simulink model "ASM_Traffic_new"  (R2024a)
settings: Solver=ode1  StartTime=SIM.tstart.v  StopTime=SIM.tend.v  FixedStep=SIM.StepSize.v  RelTol=1e-3
PostLoadFcn:
  | if any(exist('dsrtsu_mdlpostloadfcn', 'file') ~= 0), dsrtsu_mdlpostloadfcn('Execute', bdroot); end
  | try, asm_mdl_postloadfcn(bdroot, 'UpdateModel', 3600); catch, disp(lasterr); end,
InitFcn:
  | , if any(exist('rtifpga_mdlclblib', 'file') ~= 0), rtifpga_mdlclblib('Init', bdroot); end,
  | , if any(exist('dsmpb_private', 'file') ~= 0), dsmpb_private('dsmpb_mdlclblib', 'Init', bdroot); end,
undefined symbols (not defined in the file): _to_, a0b2, ASM_BrakeHydraulics_DemoSystems, ASM_VehicleDynamics_DemoSystems, b98103fe8ad365046cd0, BrakeCircuit, CPT, Crankshaft, DiscIntNeverNeededParam, dsmsi, FinalDriveAssembly, MDL, ModeSignals, Pos_BrakePedal_Maneuver, rad, RefSignals, s_to_rpm, SIM, SoftECU, Suspension, Tire, Transmission
libraries: ASM_Traffic_lib x135, simulink x100, ASM_Utils_lib x77, ASM_VehicleDynamics_lib x70, ASM_Environment_lib x22, dsmpblib x20, dsmsilib x15, MDLD_Utils_lib x10, ASM_BrakeHydraulics_lib x3
(part 27 of 63)

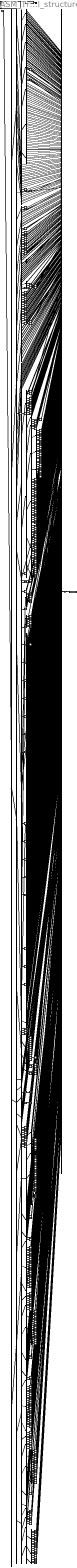
== system ASM_Traffic_new/Environment/SignalInterface/ASMSignalInterface/signal_structure ==
  ASMSignalBus : Inport
  Ambient : BusSelector  OutputSignals=T_Ambient[degC],p_Ambient[Pa]
  Angle_Fellows[x;y;z][deg] : BusSelector  OutputSignals=Angle_Roll_Fellows[deg],Angle_Pitch_Fellows[deg],Angle_Yaw_Fellows[deg],Angle_Wheel_Fellows[deg]
  BusSelector_1 : BusSelector  OutputSignals=Maneuver,Road,Traffic,GroundTruth,Sensors
  Collision_Sensor : BusSelector  OutputSignals=Collision_Sensor_1
  Collision_Sensor_1 : BusSelector  OutputSignals=Info,SensorOutput
  Common : BusSelector  OutputSignals=LaneID_PrefLane[],LaneID_Absolute[],LaneDirection_Absolute[],LaneDirection_Relative[],LaneWidth[m],LaneCurvature[1|m],Curvature[1|m]
  ContentID : Constant  Value=546881520
  Control : BusSelector  OutputSignals=Quadrant_Def_Mode[1Internal|2External],Quadrant_Dim_x[m],Quadrant_Dim_y[m],Interface_Mode[0Off|1ObjOnly|2ObjAndLanes],Interface_Init[0Off|1On],Interface_Init_Ready[0Off|1On]
  Control1 : BusSelector  OutputSignals=Quadrant_Def_Mode[1Internal|2External],Quadrant_Dim_x[m],Quadrant_Dim_y[m],Interface_Mode[0Off|1ObjOnly|2ObjAndLanes],Interface_Init[0Off|1On],Interface_Init_Ready[0Off|1On]
  CurrentLane : BusSelector  OutputSignals=Common,LeftSide,RightSide
  CustomPoints : BusSelector  OutputSignals=ID[],Object_ID[],Dist_CoorSys_S[m],Angle_Hor_CoorSys_S[deg],Pos_CoorSys_E[x;y;z][m]
  CustomPoints1 : BusSelector  OutputSignals=ID[],Object_ID[],Dist_CoorSys_S[m],Angle_Hor_CoorSys_S[deg],Pos_CoorSys_E[x;y;z][m]
  Data : BusSelector  OutputSignals=GroundTruth_Interface_Data[],HostVehicle_Data
  DataTypeConversion_{102,155..157,188,220,310..311,587,591..592,595..596,604..605} (15 alike) : DataTypeConversion  OutDataTypeStr=double
  Data_Access : BusSelector  OutputSignals=Num_MovObj[],Num_MovObj_in_GT_Area[],Num_StatObj[],Num_StatObj_in_GT_Area[],Num_Laneboundaries[],Num_Lanes[],Num_TrfLights[],Num_TrfLights_in_GT_Area[],Num_TrfSigns[],Num_TrfSigns_in_GT_Area[]
  DiscreteObjects : BusSelector  OutputSignals=Flag_DiscreteObject_Init_Ready[0|1],DiscreteObjectsState[],Data_Valid[],DiscreteObject_Data[]
  Dist_Response_Maneuver : BusSelector  OutputSignals=Distance_xy[m],Distance_z[m]
  Dist_Response_Traffic : BusSelector  OutputSignals=Distance_xy[m],Distance_z[m]
  DriverMonitoring : BusSelector  OutputSignals=DriverGazeLocation[],DriverAnimation[],DriverLizardOwlRatio[]
  FellowParameters : BusSelector  OutputSignals=Info,Data_Valid_Fellows[0|1],PosVec_MainPnt_Fellows[x;y;z][m],Length_Fellows[m],Width_Fellows[m],Height_Fellows[m],Wheel_Radius_Fellows[m],TrackWidth_Front_Fellows[m],TrackWidth_Rear_Fellows[m],WheelBase_Fellows[m],TrafficObject_Type_Fellows[],Movement_Characteristics[],Hitch_Dist[m]
  FellowSignalLabels : BusSelector  OutputSignals=d_Total_Fellows[m],LaneIdx_Total_Fellows[],s_Fellows[m],v_Fellows[km|h]
  GroundTruth : BusSelector  OutputSignals=Control,Info,Data,Data_Access,OpenSimulationInterface
  Info : BusSelector  OutputSignals=CurrentSegment[],t_local[s],s_local[m],ManeuverTime[s],ManeuverState[],ErrorFlag[],CurrentSequence[]
  Info1 : BusSelector  OutputSignals=TrafficState[],ErrorFlag[],CurrentSequence_Fellows[],CurrentSegment_Fellows[],t_local_Fellows[s],CurrentSequence_UserSignals[],CurrentSegment_UserSignals[],t_local_UserSignals[s],CurrentSegment[],t_local[s]
  Info2 : BusSelector  OutputSignals=FellowParameters_Sfcn_State[],FellowParameters_Data_Valid[0|1]
  Info3 : BusSelector  OutputSignals=Interface_State[]
  Info4 : BusSelector  OutputSignals=Sfunc_State[],Data_Valid[0|1],Flag_Sensor_Init_Ready[0|1]
  Info5 : BusSelector  OutputSignals=TrafficSignSensor_Dyn_Sfcn_State[],TrafficSignSensor_Dyn_Data_Valid[0|1]
  Info6 : BusSelector  OutputSignals=Flag_Object_In_Scope[0Out|1In],Flag_Sensor_Apex_In_Object[0Out|1In],ObjectSensor3D_Sfcn_State[],ObjectSensor3D_Data_Valid[0|1],Flag_Sensor_Init_Ready[0|1]
  Info7 : BusSelector  OutputSignals=Flag_Object_In_Scope[0Out|1In],Flag_Sensor_Apex_In_Object[0Out|1In],ObjectSensor3D_Sfcn_State[],ObjectSensor3D_Data_Valid[0|1],Flag_Sensor_Init_Ready[0|1]
  Info8 : BusSelector  OutputSignals=ObjectSensor2D_Sfcn_State[],ObjectSensor2D_Data_Valid[0|1],Flag_Sensor_Init_Ready[0|1]
  InfoBlock : Subsystem
      mask Display: fprintf('Structural changes of the signal bus require an update \nof the ''ASMSignalCollector'' block. \n\nTo start the update process double click the parent block.\n\n WARNING:\n During update this subsystem will be cleared completely')
  InitialVehStates : BusSelector  OutputSignals=s_Vehicle_Init[m],d_Vehicle_Init[m],LaneIdx_Vehicle_Init[],Pos_z_Vehicle_Rel_Init[m],Angle_Yaw_Vehicle_Rel_Init[deg],v_Vehicle_Init[km|h],Route_Id_Init[],Route_Direction_Init[]
  LaneSensor_Dynamic : BusSelector  OutputSignals=Parameters,Sensor_Output
  Lane_Network : BusSelector  OutputSignals=LaneNetwork_State[],Data_Valid[],LaneNetwork_Data[]
  Lanes_Left : BusSelector  OutputSignals=LaneID_PrefLane[],LaneID_Absolute[],LaneDirection_Absolute[],LaneDirection_Relative[],LaneWidth[m],LaneCurvature[1|m],Pos_Left[x;y;z][m],Yaw_Angle_Left[deg],Yaw_Angle_RelVehicle_Left[deg],Curvature_Left[1|m],MarkerType_Left[],MarkerWidth_Left[m],MarkerColor_Left[],LineID_1_Left[],LineID_2_Left[],Distance_Marker_Left[m],Pos_Right[x;y;z][m],Yaw_Angle_Right[deg],Yaw_Angle_RelVehicle_Right[deg],Curvature_Right[1|m],MarkerType_Right[],MarkerWidth_Right[m],MarkerColor_Right[],LineID_1_Right[],LineID_2_Right[],Distance_Marker_Right[m]
  Lanes_Right : BusSelector  OutputSignals=LaneID_PrefLane[],LaneID_Absolute[],LaneDirection_Absolute[],LaneDirection_Relative[],LaneWidth[m],LaneCurvature[1|m],Pos_Left[x;y;z][m],Yaw_Angle_Left[deg],Yaw_Angle_RelVehicle_Left[deg],Curvature_Left[1|m],MarkerType_Left[],MarkerWidth_Left[m],MarkerColor_Left[],LineID_1_Left[],LineID_2_Left[],Distance_Marker_Left[m],Pos_Right[x;y;z][m],Yaw_Angle_Right[deg],Yaw_Angle_RelVehicle_Right[deg],Curvature_Right[1|m],MarkerType_Right[],MarkerWidth_Right[m],MarkerColor_Right[],LineID_1_Right[],LineID_2_Right[],Distance_Marker_Right[m]
  LeftSide : BusSelector  OutputSignals=Pos_Left[x;y;z][m],Yaw_Angle_Left[deg],Yaw_Angle_RelVehicle_Left[deg],Curvature_Left[1|m],MarkerType_Left[],MarkerWidth_Left[m],MarkerColor_Left[],LineID_1_Left[],LineID_2_Left[],Distance_Marker_Left[m]
  Line_Sensor_Data : BusSelector  OutputSignals=RoadNetworkData
  MDLD_DATA_CAPTURE : MDLD_Utils_lib/ModelDeskPlotInterface/DataCapture_Sfcn/MDLD_DATA_CAPTURE  inputPortWidth=12543  measurementSignals=[0 0 0 0 0 0 0 0 0 0 0 0 0 0 0 0 0 0 0 0 0 0 0 0 0 0 0 0 0 0 0 0 0 0 0 0 0 0 0 0 0 0 0 0 0 0 0 0 0 0 0 0 0 0 0 0 0 0 0 0 0 0 0 0 0 0 0 0 0 0 0 0 0 0 0 0 0 0 0 0 0 0 0 0 0 0 0 0 0 0 0 0 0 0 0 0 0 0 0 0 0 0 0 0 0 0 0 0 0 0 0 0 0 0 0 0 0 0 0 0 0 0 0 0 0 0 0 0 0 0 0 0 0 0 0 0 0 0 0 0 0 0 0 0 0 0 0 0 0 0 0 0 0 0 0 0 0 0 0 0 0 0 0 0 0 0 0 0 0 0 0 0 0 0 0 0 0 0 0 0 0 0 0 0 0 0 0 0 0 0 0 0 0 0 0 0 0 0 0 0 0 0 0 0 0 0 0 0 0 0 0 0 0 0 0 0 0 0 0 0 0 0 0 0 0 0 0 0 0 0 0 0 0 0 0 0 0 0 0 0 0 0 0 0 0 0 0 0 0 0 0 0 0 0 0 0 0 0 0 0 0 0 0 0 0 0 0 0 0 0 0 0 0 0 0 0 0 0 0 0 0 0 0 0 0 0 0 0 0 0 0 0 0 0 0 0 0 0 0 0 0 0 0 0 0 0 0 0 0 0 0 0 0 0 0 0 0 0 0 0 0 0 0 0 0 0 0 0 0 0 0 0 0 0 0 0 0 0 0 0 0 0 0 0 0 0 0 0 0 0 0 0 0 0 0 0 0 0 0 0 0 0 0 0 0 0 0 0 0 0 0 0 0 0 0 0 0 0 0 0 0 0 0 0 0 0 0 0 0 0 0 0 0 0 0 0 0 0 0 0 0 0 0 0 0 0 0 0 0 0 0 0 0 0 0 0 0 0 0 0 0 0 0 0 0 0 0 0 0 0 0 0 0 0 0 0 0 0 0 0 0 0 0 0 0 0 0 0 0 0 0 0 0 0 0 0 0 0 0 0 0 0 0 0 0 0 0 0 0 0 0 0 0 0 0 0 0 0 0 0 0 0 0 0 0 0 0 0 0 0 0 0 0 0 0 0 0 0 0 0 0 0 0 0 0 0 0 0 0 0 0 0 0 0 0 0 0 0 0 0 0 0 0 0 0 0 0 0 0 0 0 0 0 0 0 0 0 0 0 0 0 0 0 0 0 0 0 0 0 0 0 0 0 0 0 0 0 0 0 0 0 0 0 0 0 0 0 0 0 0 0 0 0 0 0 0 0 0 0 0 0 0 0 0 0 0 0 0 0 0 0 0 0 0 0 0 0 0 0 0 0 0 0 0 0 0 0 0 0 0 0 0 0 0 0 0 0 0 0 0 0 0 0 0 0 0 0 0 0 0 0 0 0 0 0 0 0 0 0 0 0 0 0 0 0 0 0 0 0 0 0 0 0 0 0 0 0 0 0 0 0 0 0 0 0 0 0 0 0 0 0 0 0 0 0 0 0 0 0 0 0 0 0 0 0 0 0 0 0 0 0 0 0 0 0 0 0 0 0 0 0 0 0 0 0 0 0 0 0 0 0 0 0 0 0 0 0 0 0 0 0 0 0 0 0 0 0 0 0 0 0 0 0 0 0 0 0 0 0 0 0 0 0 0 0 0 0 0 0 0 0 0 0 0 0 0 0 0 0 0 0 0 0 0 0 0 0 0 0 0 0 0 0 0 0 0 0 0 0 0 0 0 0 0 0 0 0 0 0 0 0 0 0 0 0 0 0 0 0 0 0 0 0 0 0 0 0 0 0 0 0 0 0 0 0 0 0 0 0 0 0 0 0 0 0 0 0 0 0 0 0 0 0 0 0 0 0 0 0 0 0 0 0 0 0 0 0 0 0 0 0 0 0 0 0 0 0 0 0 0 0 0 0 0 0 0 0 0 0 0 0 0 0 0 0 0 0 0 0 0 0 0 0 0 0 0 0 0 0 0 0 0 0 0 0 0 0 0 0 0 0 0 0 0 0 0 0 0 0 0 0 0 0 0 0 0 0 0 0 0 0 0 0 0 0 0 0 0 0 0 0 0 0 0 0 0 0 0 0 0 0 0 0 0 0 0 0 0 0 0 0 0 0 0 0 0 0 0 0 0 0 0 0 0 0 0 0 0 0 0 0 0 0 0 0 0 0 0 0 0 0 0 0 0 0 0 0 0 0 0 0 0 0 0 0 0 0 0 0 0 0 0 0 0 0 0 0 0 0 0 0 0 0 0 0 0 0 0 0 0 0 0 0 0 0 0 0 0 0 0 0 0 0 0 0 0 0 0 0 0 0 0 0 0 0 0 0 0 0 0 0 0 0 0 0 0 0 0 0 0 0 0 0 0 0 0 0 0 0 0 0 0 0 0 0 0 0 0 0 0 0 0 0 0 0 0 0 0 0 0 0 0 0 0 0 0 0 0 0 0 0 0 0 0 0 0 0 0 0 0 0 0 0 0 0 0 0 0 0 0 0 0 0 0 0 0 0 0 0 0 0 0 0 0 0 0 0 0 0 0 0 0 0 0 0 0 0 0 0 0 0 0 0 0 0 0 0 0 0 0 0 0 0 0 0 0 0 0 0 0 0 0 0 0 0 0 0 0 0 0 0 0 0 0 0 0 0 0 0 0 0 0 0 0 0 0 0 0 0 0 0 0 0 0 0 0 0 0 0 0 0 0 0 0 0 0 0 0 0 0 0 0 0 0 0 0 0 0 0 0 0 0 0 0 0 0 0 0 0 0 0 0 0 0 0 0 0 0 0 0 0 0 0 0 0 0 0 0 0 0 0 0 0 0 0 0 0 0 0 0 0 0 0 0 0 0 0 0 0 0 0 0 0 0 0 0 0 0 0 0 0 0 0 0 0 0 0 0 0 0 0 0 0 0 0 0 0 0 0 0 0 0 0 0 0 0 0 0 0 0 0 0 0 0 0 0 0 0 0 0 0 0 0 0 0 0 0 0 0 0 0 0 0 0 0 0 0 0 0 0 0 0 0 0 0 0 0 0 0 0 0 0 0 0 0 0 0 0 0 0 0 0 0 0 0 0 0 0 0 0 0 0 0 0 0 0 0 0 0 0 0 0 0 0 0 0 0 0 0 0 0 0 0 0 0 0 0 0 0 0 0 0 0 0 0 0 0 0 0 0 0 0 0 0 0 0 0 0 0 0 0 0 0 0 0 0 0 0 0 0 0 0 0 0 0 0 0 0 0 0 0 0 0 0 0 0 0 0 0 0 0 0 0 0 0 0 0 0 0 0 0 0 0 0 0 0 0 0 0 0 0 0 0 0 0 0 0 0 0 0 0 0 0 0 0 0 0 0 0 0 0 0 0 0 0 0 0 0 0 0 0 0 0 0 0 0 0 0 0 0 0 0 0 0 0 0 0 0 0 0 0 0 0 0 0 0 0 0 0 0 0 0 0 0 0 0 0 0 0 0 0 0 0 0 0 0 0 0 0 0 0 0 0 0 0 0 0 0 0 0 0 0 0 0 0 0 0 0 0 0 0 0 0 0 0 0 0 0 0 0 0 0 0 0 0 0 0 0 0 0 0 0 0 0 0 0 0 0 0 0 0 0 0 0 0 0 0 0 0 0 0 0 0 0 0 0 0 0 0 0 0 0 0 0 0 0 0 0 0 0 0 0 0 0 0 0 0 0 0 0 0 0 0 0 0 0 0 0 0 0 0 0 0 0 0 0 0 0 0 0 0 0 0 0 0 0 0 0 0 0 0 0 0 0 0 0 0 0 0 0 0 0 0 0 0 0 0 0 0 0 0 0 0 0 0 0 0 0 0 0 0 0 0 0 0 0 0 0 0 0 0 0 0 0 0 0 0 0 0 0 0 0 0 0 0 0 0 0 0 0 0 0 0 0 0 0 0 0 0 0 0 0 0 0 0 0 0 0 0 0 0 0 0 0 0 0 0 0 0 0 0 0 0 0 0 0 0 0 0 0 0 0 0 0 0 0 0 0 0 0 0 0 0 0 0 0 0 0 0 0 0 0 0 0 0 0 0 0 0 0 0 0 0 0 0 0 0 0 0 0 0 0 0 0 0 0 0 0 0 0 0 0 0 0 0 0 0 0 0 0 0 0 0 0 0 0 0 0 0 0 0 0 0 0 0 0 0 0 0 0 0 0 0 0 0 0 0 0 0 0 0 0 0 0 0 0 0 0 0 0 0 0 0 0 0 0 0 0 0 0 0 0 0 0 0 0 0 0 0 0 0 0 0 0 0 0 0 0 0 0 0 0 0 0 0 0 0 0 0 0 0 0 0 0 0 0 0 0 0 0 0 0 0 0 0 0 0 0 0 0 0 0 0 0 0 0 0 0 0 0 0 0 0 0 0 0 0 0 0 0 0 0 0 0 0 0 0 0 0 0 0 0 0 0 0 0 0 0 0 0 0 0 0 0 0 0 0 0 0 0 0 0 0 0 0 0 0 0 0 ...(+21088 chars)]  downsampling=1  samplingPeriod=SIM.StepSize.v  uuid=0  ASMProperties=struct('Name','mdld_data_capture','Version','1.0','Library','mdld_utils_lib')  startTriggerDelay=0  startTriggerLogic=0  startTriggerCount=0  startTriggerConditions=[0,0,0,0,0,0,0,0,0]  stopTriggerDelay=0  stopTriggerLogic=0  stopTriggerCount=0  stopTriggerConditions=[0,0,0,0,0,0,0,0,0]  ContentID_RefStruct=546881520
  Maneuver : BusSelector  OutputSignals=ManeuverScheduler,UserSignals_Customized,VehicleInitStates,Testbench,ParkingBrake,StartButton,Sw_TipShift[-1Down|0Off|1Up]
  ManeuverScheduler : BusSelector  OutputSignals=MdlControl,InitialVehStates,ModeSignals,RefSignals,Parameters,UserSignals,Info
  MdlControl : BusSelector  OutputSignals=Reset_VehicleStates[0|1],RoadControl[],Get_VehPos_Trigger[],Keep_VehiclePosition[0|1]
  Measurement_Points : BusSelector  OutputSignals=Distance_MeasPnt_Marker_Left[m],Distance_MeasPnt_Marker_Right[m],Velocity_MeasPnt_Marker_Left[m|s],Velocity_MeasPnt_Marker_Right[m|s]
  ModeSignals : BusSelector  OutputSignals=Mode_AccBr[1Stim|2Driver],Mode_GearClutch[1Stim|2Driver|3OpenClutch|4RefGear],Mode_Steer[1Stim|2Driver|3Fix],Mode_Road[1NoRoad|2Straight|3Circle|4Road],LatDriver[1LatCtrl1|2LatCtrl2],Mode_LatCtrl[1Pos|2Yaw],Mode_AdaptVelocityToRoad[1Off|2On],Mode_ForceToRoad[1Off|2On],Mode_SelectorLever[1Stim|2Driver],Mode_CurvatureCalculation[1Road|2Driver],Mode_TrafficDriver[1Off|2On],Mode_RelativeLane[0CenterLane|1PreferredLane]
  Network_Item : BusSelector  OutputSignals=Network_Item_ID[],Network_Item_Type[],Network_Item_Type_Absolute[],Preferred_Lane_Direct[],Preferred_Lane_Oncoming[]
  ObjectData : BusSelector  OutputSignals=Object_Positions,Object_Properties_Box,Object_Custom_Values
  ObjectData1 : BusSelector  OutputSignals=Object_Positions,Object_Properties_Box,Object_Custom_Values
  ObjectData2 : BusSelector  OutputSignals=Object_Positions,Object_Properties_Box,Object_Custom_Values
  ObjectParameters : BusSelector  OutputSignals=FellowParameters,TrafficObjects,DiscreteObjects
  Object_Custom_Values : BusSelector  OutputSignals=Object_Valid[0|1],CustomValues[]
  Object_Custom_Values1 : BusSelector  OutputSignals=Object_Valid[0|1],CustomValues[]
  Object_Custom_Values2 : BusSelector  OutputSignals=Object_Valid[0|1],CustomValues[]
  Object_Positions : BusSelector  OutputSignals=Pos_x_MainPnt_Objects_CoorSysE[m],Pos_y_MainPnt_Objects_CoorSysE[m],Pos_z_MainPnt_Objects_CoorSysE[m],Angle_x_Objects_CoorSysE[deg],Angle_y_Objects_CoorSysE[deg],Angle_z_Objects_CoorSysE[deg],Network_Item_Type[],Network_Item_Id[],Object_ID[]
  Object_Positions1 : BusSelector  OutputSignals=Pos_x_MainPnt_Objects_CoorSysE[m],Pos_y_MainPnt_Objects_CoorSysE[m],Pos_z_MainPnt_Objects_CoorSysE[m],Angle_x_Objects_CoorSysE[deg],Angle_y_Objects_CoorSysE[deg],Angle_z_Objects_CoorSysE[deg],Network_Item_Type[],Network_Item_Id[],Object_ID[]
  Object_Positions2 : BusSelector  OutputSignals=Pos_x_MainPnt_Objects_CoorSysE[m],Pos_y_MainPnt_Objects_CoorSysE[m],Pos_z_MainPnt_Objects_CoorSysE[m],Angle_x_Objects_CoorSysE[deg],Angle_y_Objects_CoorSysE[deg],Angle_z_Objects_CoorSysE[deg],Network_Item_Type[],Network_Item_Id[],Object_ID[]
  Object_Properties_Box : BusSelector  OutputSignals=Flag_BoxProperties[0|1],PosVec_x_CenterPnt_Object[m],PosVec_y_CenterPnt_Object[m],PosVec_z_CenterPnt_Object[m],Length_Object[m],Width_Object[m],Height_Object[m],Object_Type[]
  Object_Properties_Box1 : BusSelector  OutputSignals=Flag_BoxProperties[0|1],PosVec_x_CenterPnt_Object[m],PosVec_y_CenterPnt_Object[m],PosVec_z_CenterPnt_Object[m],Length_Object[m],Width_Object[m],Height_Object[m],Object_Type[]
  Object_Properties_Box2 : BusSelector  OutputSignals=Flag_BoxProperties[0|1],PosVec_x_CenterPnt_Object[m],PosVec_y_CenterPnt_Object[m],PosVec_z_CenterPnt_Object[m],Length_Object[m],Width_Object[m],Height_Object[m],Object_Type[]
  Object_Sensor_2D_1 : BusSelector  OutputSignals=Parameters,SensorIndex,SensorStatus,SensorOutput,Info,ObjectData
  Object_Sensor_3D_1 : BusSelector  OutputSignals=Parameter,SensorIndex,Info,SensorOutput,SensorTimeStamp,RadarEffects,CustomPoints,ObjectData
  Object_Sensor_3D_2 : BusSelector  OutputSignals=Parameter,SensorIndex,Info,SensorOutput,SensorTimeStamp,RadarEffects,CustomPoints,ObjectData
  OpenSimulationInterface : BusSelector  OutputSignals=MovObj_Type[],MovObj_Vehicle_Type[],MovObj_ID[],MovObj_Position_x[m],MovObj_Position_y[m],MovObj_Position_z[m],MovObj_Orientation_x[deg],MovObj_Orientation_y[deg],MovObj_Orientation_z[deg],MovObj_Length[m],MovObj_Width[m],MovObj_Height[m]
  Parameter : BusSelector  OutputSignals=Sensor_Enable[0Off|1On],SensorIdx[],t_Offs_Sensor[s],t_Cycle_Sensor[s],t_Delay_SensorOutput[s],Geometry[],Pos_Sensor_Apex_CoorSys_V[x;y;z][m],Angle_Orientation_Sensor_CoorSys_V[x;y;z][deg],Length_ScopeZone[m],Angle_ScopeZone_Horizontal[deg],Angle_ScopeZone_Vertical[deg],Length_ScopeZone_Head[m],Length_BlindZone[m],Occlusion_Mode[1No_Occlusion|2Basic_3D|3Occlusion_Ratio_3D],Threshold_Occlusion_Ratio[0_1],Object_Points_Calculation_Enable[0Off|1On],Object_Points_Occlusion_Enable[0Off|1On]
  Parameter1 : BusSelector  OutputSignals=Sensor_Enable[0Off|1On],SensorIdx[],t_Offs_Sensor[s],t_Cycle_Sensor[s],t_Delay_SensorOutput[s],Geometry[],Pos_Sensor_Apex_CoorSys_V[x;y;z][m],Angle_Orientation_Sensor_CoorSys_V[x;y;z][deg],Length_ScopeZone[m],Angle_ScopeZone_Horizontal[deg],Angle_ScopeZone_Vertical[deg],Length_ScopeZone_Head[m],Length_BlindZone[m],Occlusion_Mode[1No_Occlusion|2Basic_3D|3Occlusion_Ratio_3D],Threshold_Occlusion_Ratio[0_1],Object_Points_Calculation_Enable[0Off|1On],Object_Points_Occlusion_Enable[0Off|1On]
  Parameters : BusSelector  OutputSignals=a_x_Max[m|s2],a_x_Brake_Threshold[m|s2],a_y_Max[m|s2],Curv_Road_Circle[1|m],Gear_Max[],Width_Deadzone_LatCtrl[m],v_Lat[m|s],Object_Type_ID[],Driver_Type_Index[]
  Parameters1 : BusSelector  OutputSignals=Enable_Evaluation[0|1],Evaluation_Distance[m],Border_Mode[0Center|1Inner|2Outer],Enable_Junction_Evaluation[0|1],Num_Lanes[Left;Right],Enable_MeasPoint[0|1],MeasPoint_1_CoorSysV[x;y][m],MeasPoint_2_CoorSysV[x;y][m],MeasPoint_3_CoorSysV[x;y][m],MeasPoint_4_CoorSysV[x;y][m],MeasPoint_1_CoorSysE[x;y][m],MeasPoint_2_CoorSysE[x;y][m],MeasPoint_3_CoorSysE[x;y][m],MeasPoint_4_CoorSysE[x;y][m]
  Parameters2 : BusSelector  OutputSignals=Sensor_Enable[0Off|1On],Pos_Sensor_Apex_CoorSys_V[x;y;z][m],Angle_Orientation_Sensor_CoorSys_V[x;y;z][deg],Length_ScopeZone[m],Angle_ScopeZone_Horizontal[deg],Angle_ScopeZone_Vertical[deg],Angle_Sign_Orientation_Max[deg]
  Parameters3 : BusSelector  OutputSignals=Sensor_Enable[0Off|1On],SensorIdx[],t_Offs_Sensor[s],t_Cycle_Sensor[s],t_Delay_SensorOutput[s],Pos_Sensor_Apex_CoorSys_V[x;y;z][m],Angle_z_Orientation_Sensor_CoorSys_V[deg],Angle_ScopeZone_Horizontal[deg],Length_ScopeZone[m],Num_SensorRays_Used[],Sensor_Detection_Mode[1Ray|2Sector],Object_Detection_Mode[1Object|2Continuous|3All]
  ParkingBrake : BusSelector  OutputSignals=Sw_ParkingBrake[0Off|1On]
  Pos_Fellows_MainPnt_CoorSys_E[x;y;z][m] : BusSelector  OutputSignals=Pos_x_Fellows[m],Pos_y_Fellows[m],Pos_z_Fellows[m]
  Pos_Vehicle_GPS[Long;Lat][deg] : BusSelector  OutputSignals=Longitude[deg],Latitude[deg],Heading[deg]
  RadarEffects : BusSelector  OutputSignals=ID[],Object_ID[],Dist_CoorSys_S[m],Angle_Hor_CoorSys_S[deg],Pos_ObjectPoint_CoorSys_E[x;y;z][m]
  RadarEffects1 : BusSelector  OutputSignals=ID[],Object_ID[],Dist_CoorSys_S[m],Angle_Hor_CoorSys_S[deg],Pos_ObjectPoint_CoorSys_E[x;y;z][m]
  RefSignals : BusSelector  OutputSignals=Pos_AccPedal_Maneuver[%],Pos_BrakePedal_Maneuver[%],Pos_ClutchPedal_Maneuver[%],Gear_Maneuver[],Angle_SteeringWheel_Maneuver[deg],v_Vehicle_Ref_Maneuver[m|s],v_Vehicle_Ref_Maneuver[km|h],d_Maneuver[m],LaneIdx_Maneuver[],Dist_Def_Maneuver[],v_Vehicle_Ref_Preview_Maneuver[m|s],v_Vehicle_Ref_Preview_State[0Invalid|1CurrentSeg|2NextSeg],Sw_SteeringMode_Maneuver[1Angle|2Trq],Trq_Steering_Maneuver[Nm],SelectorLever_Maneuver[],Dist_Def_Refline_Maneuver[]
  Reshape_{34,40,101,111..112,123,125..137,154..177,188,204..205,208..217,221..308,311..322,327..332,335..349,354,571..574,577..588,592,596,604..605,616..627,633..639,642..662,664..665,676..677,688..689,693..716,719..747,754..755,766..767,771..794,797..825,831,841..848,852..870} (382 alike) : Reshape
  RightSide : BusSelector  OutputSignals=Pos_Right[x;y;z][m],Yaw_Angle_Right[deg],Yaw_Angle_RelVehicle_Right[deg],Curvature_Right[1|m],MarkerType_Right[],MarkerWidth_Right[m],MarkerColor_Right[],LineID_1_Right[],LineID_2_Right[],Distance_Marker_Right[m]
  Road : BusSelector  OutputSignals=Road_Init,Road_ASMVeh,Road_ContactPoints,Road_Preview,Road_Info,Road_TrafficFellows,UserSignals,TrafficObject_Data[],UserSignals_Customized,Pos_Vehicle_GPS[Long;Lat][deg],Ambient,LaneSensor_Dynamic,Lane_Network
  Road_ASMVeh : BusSelector  OutputSignals=s_Veh_Road[m],s_Total_Veh_Road[m],d_Total_Veh_Road[m],s_Veh_Road_Trj[m],LaneIdx_Total_Veh_Road[],Curv_Veh_Road[1|m],Pos_x_Ref_Veh_Road[m],Pos_y_Ref_Veh_Road[m],Angle_Yaw_Veh_Road[deg],Slope_Veh_Road[%],v_Wind_Coor_Sys_E[x;y;z][m|s],Slope_Lateral_Veh_Road[deg]
  Road_ContactPoints : BusSelector  OutputSignals=Pos_z_CP[:][m],Fric_Coeff_CP[:][],UnitVec_z_CP[:][x;y;z],Sw_Tire_Parameter_Set_CP[:][1|2|3|4]
  Road_Info : BusSelector  OutputSignals=RoadState[],RouteLength_Veh[m],Flag_RouteClosed_Veh[0|1],Dist_Response_Maneuver,Speed_Limit_Veh[km|h],Network_Item_Type_Veh[],Network_Item_Id_Veh[],RoadSegment_Veh[],LaneSection_Veh[],RoadWidth_Veh[m],Network_Load_Idx[],d_Veh_Ref_Line[m],Dist_Border_Left[m],Dist_Border_Right[m],Trf_Driver_Data,Line_Sensor_Data,V2X_Data[]
  Road_Init : BusSelector  OutputSignals=Pos_Vehicle_Init_CoorSys_E[x;y;z][m],Angle_Vehicle_Init_CoorSys_E[x;y;z][rad]
  Road_Preview : BusSelector  OutputSignals=Pos_x_Preview_Road[m],Pos_y_Preview_Road[m],Curv_Preview_Road[1|m],Speed_Limit_Preview_Road[km|h],Pos_z_Preview_Road[m],Roll_Preview_Road[deg],Pitch_Preview_Road[deg],x_Preview_DriverCurv[m],y_Preview_DriverCurv[m]
  Road_TrafficFellows : BusSelector  OutputSignals=Pos_x_Fellows_Road[m],Pos_y_Fellows_Road[m],Pos_z_Fellows_Road[m],Angle_Yaw_Fellows_Road[deg],Angle_Pitch_Fellows_Road[deg],Angle_Roll_Fellows_Road[deg],Curv_Fellows_Road[1|m],d_Total_Fellows_Road[m],LaneIdx_Total_Fellows_Road[],RoadSegment_Fellows[],LaneSection_Fellows[],Speed_Limit_Fellows[],Network_Item_Type_Fellows[],Network_Item_Id_Fellows[],d_Fellows_RefLine[m],RouteLength_Fellows[m],Flag_RouteClosed_Fellows[0|1],Dist_Response_Traffic,Angle_Yaw_Fellows_RoadRefline[deg]
  SFunction_Info : BusSelector  OutputSignals=Sfcn_State[0|1],Input_Data_Valid[0|1],Data_Valid[0|1]
  SensorIndex : BusSelector  OutputSignals=Idx_Sensor[]
  SensorIndex1 : BusSelector  OutputSignals=Idx_Sensor[]
  SensorIndex2 : BusSelector  OutputSignals=Idx_Sensor[]
  SensorOutput : BusSelector  OutputSignals=Collision_Flag[0NoCollision|1Collision],Collision_Flag_Held[0NoCollision|1Collision],Object_ID[],Time_Collision[s],Pos_Collision_Point[x;y][m],v_Collision_CoG_Vehicle[x;y][m|s],v_Collision_CoG_Vehicle_Total[m|s],v_Rel_Collision_Point[x;y][m|s],v_Rel_Collision_Point_Total[m|s]
  SensorOutput1 : BusSelector  OutputSignals=v_Rel_Object[m|s],v_Object_CoorSys_S[x;y;z][m|s],a_Rel_Object[m|s2],a_Object_CoorSys_S[x;y;z][m|s2],Dist_Object[m],Angle_Hor_Object[deg],Angle_Ver_Object[deg],Pos_Sensor_Apex_E[x;y;z][m],Pos_Object_NearestPnt_S[x;y;z][m],Pos_Object_NearestPnt_E[x;y;z][m],Object_Info[-1None|1Fellow|2Static],Object_ID[],Object_Type[],Object_Age[s],Object_In_Scope_Entry_First[s],Object_In_Scope_Entry_Number[],Occlusion_Ratio_Object[-1|0_1],Flag_NearestPnt_Occluded[-1|0|1],Pos_NearestSurf_Pnt1_CoorSys_S[x;y;z][m],Pos_NearestSurf_Pnt2_CoorSys_S[x;y;z][m],Pos_NearestSurf_Pnt3_CoorSys_S[x;y;z][m],Pos_NearestSurf_Pnt4_CoorSys_S[x;y;z][m],NearestSurf_Pnts_Index[],NearestSurf_Index[]
  SensorOutput2 : BusSelector  OutputSignals=v_Rel_Object[m|s],v_Object_CoorSys_S[x;y;z][m|s],a_Rel_Object[m|s2],a_Object_CoorSys_S[x;y;z][m|s2],Dist_Object[m],Angle_Hor_Object[deg],Angle_Ver_Object[deg],Pos_Sensor_Apex_E[x;y;z][m],Pos_Object_NearestPnt_S[x;y;z][m],Pos_Object_NearestPnt_E[x;y;z][m],Object_Info[-1None|1Fellow|2Static],Object_ID[],Object_Type[],Object_Age[s],Object_In_Scope_Entry_First[s],Object_In_Scope_Entry_Number[],Occlusion_Ratio_Object[-1|0_1],Flag_NearestPnt_Occluded[-1|0|1],Pos_NearestSurf_Pnt1_CoorSys_S[x;y;z][m],Pos_NearestSurf_Pnt2_CoorSys_S[x;y;z][m],Pos_NearestSurf_Pnt3_CoorSys_S[x;y;z][m],Pos_NearestSurf_Pnt4_CoorSys_S[x;y;z][m],NearestSurf_Pnts_Index[],NearestSurf_Index[]
  SensorOutput3 : BusSelector  OutputSignals=Angle_Hor_Rel[deg],Object_ID[],Object_Type[],Distance[m],v_Rel[m|s],a_Rel[m|s2],Height_Min[m],Height_Max[m]
  SensorOutput[] : BusSelector  OutputSignals=Traffic_Sign_Valid[0|1],TrafficObject_ID[],TrafficObject_Type[],Pos_CoorSys_E[x;y;z][m],Angle_CoorSys_E[x;y;z][deg],Pos_CoorSys_S[x;y;z][m],Angle_Hor_Rel[deg],Angle_Ver_Rel[deg],Angle_Sign_Orientation_Rel[deg],Distance[m],Traffic_Sign_Type[],Traffic_Sign_Subtype[],Traffic_Sign_Value[],Traffic_Sign_Country[],Traffic_Sign_Visibility[0_100],Traffic_Sign_Lanes[],Object_Stream_ID[],Object_State[],Parent_Object_ID[],Network_Item_Type[0Junction|1Road],Network_Item_ID[]
  SensorStatus : BusSelector  OutputSignals=Flag_Object_In_Scope[0Out|1In],Flag_Sensor_Apex_In_Object[0Out|1In]
  SensorTimeStamp : BusSelector  OutputSignals=ObjectSample[s],SensorCalculation[s]
  SensorTimeStamp1 : BusSelector  OutputSignals=ObjectSample[s],SensorCalculation[s]
  Sensor_Front_1 : BusSelector  OutputSignals=Info,SensorOutput[],Parameters
  Sensor_Output : BusSelector  OutputSignals=SFunction_Info,Network_Item,CurrentLane,Lanes_Left,Lanes_Right,Measurement_Points
  Sensors : BusSelector  OutputSignals=Collision_Sensor,TrafficSign_Sensor_Dyn,Object_Sensor_3D_1,Object_Sensor_3D_2,Object_Sensor_2D_1
  SignalFilter : Mux  Inputs=870
  SignalFilterGain : Gain
  StartButton : BusSelector  OutputSignals=Sw_StartButton[0Off|1On],Mode_StartButtonState[1Stim|2SoftECU],State_StartButton[-1PowerOff|0Acc|1PowerOn|2StarterOn]
  Terminator : Terminator
  Testbench : BusSelector  OutputSignals=Sw_Testbench[0Off|1On],EngOpNum[],n_Engine_Set[rpm]
  Traffic : BusSelector  OutputSignals=Traffic_Signals_toEnvironment,FellowSignalLabels,ObjectParameters
  TrafficObjects : BusSelector  OutputSignals=Flag_TrafficObject_Init_Ready[0|1],TrafficObjectsState[],Data_Valid[],TrafficObject_Type_Data[]
  TrafficSign_Sensor_Dyn : BusSelector  OutputSignals=Sensor_Front_1
  Traffic_Signals_toEnvironment : BusSelector  OutputSignals=s_Fellows_Ref_Scheduler[m],d_Fellows_Ref_Scheduler[m],v_Fellows_Ref_Scheduler[km|h],LaneIdx_Fellows_Ref_Scheduler[],RelativeLane_Mode_Fellows[0CenterLane|1PreferredLane],ForceToRoad_Fellows_Ref_Scheduler[0|1],v_Lat_Fellows_Ref_Scheduler[m|s],Direction_Fellows_Ref_Scheduler[-1|1],Route_Id_Fellows_Ref_Scheduler[],Dist_Def_Trf[],Flag_FellowUsed[0|1],a_x_Vehicle_Ref[m|s2],Dist_Refline_Response[m],Info,a_Fellows_Ref_Scheduler[m|s2],UserSignals_Fellows[],d_Total_Fellows[m],LaneIdx_Total_Fellows[],v_Fellows[km|h],Pos_Fellows_MainPnt_CoorSys_E[x;y;z][m],Angle_Fellows[x;y;z][deg],Angle_Wheel_Fellows[deg],v_Fellows[x;y;z][km|h],w_Fellows[x;y;z][deg|s],UserSignals_Customized,Control
  Trf_Driver_Data : BusSelector  OutputSignals=Route_Idx_Veh[],Route_Idx_Fellows[],RoadNetworkData
  UserSignals : BusSelector  OutputSignals=User1[],User2[],User3[],User4[],User5[],User6[],User7[],User8[],User9[],User10[],User11[],User12[],User13[],User14[],User15[],User16[],User17[],User18[],User19[],User20[],User21[],User22[],User23[],User24[],User25[],User26[],User27[],User28[],User29[],User30[]
  UserSignals1 : BusSelector  OutputSignals=User1[],User2[],User3[],User4[],User5[],User6[],User7[],User8[],User9[],User10[]
  UserSignals_Customized : BusSelector  OutputSignals=ExternalSegmentEnd_Mode[],ExternalSegmentEnd_Value[],ASM_Vehicle_TurnLights[],ECU_Commands[],Mnv_DataStream_5[],Mnv_DataStream_6[],Mnv_DataStream_7[],Mnv_DataStream_8[],Mnv_DoorFL[],Mnv_DoorFR[],Mnv_DoorRL[],Mnv_DoorRR[],Mnv_Hood[],Mnv_Trunk[]
  UserSignals_Customized1 : BusSelector  OutputSignals=GPS_Method[],Const_Offset_Lat[deg],Const_Offset_Long[deg],User4[],User5[],User6[],User7[],User8[],User9[],User10[]
  UserSignals_Customized2 : BusSelector  OutputSignals=ManeuverSegmentEndTrigger[0|1],DriverMonitoring,UserSignals,Fellow1_TurnLights,Fellow2_TurnLights,Fellow3_TurnLights,Fellow4_TurnLights,Fellow5_TurnLights,Fellow6_TurnLights,Fellow7_TurnLights,Fellow8_TurnLights,Fellow9_TurnLights,Fellow10_TurnLights,Fellow11_TurnLights,Fellow12_TurnLights,Fellow13_TurnLights,Fellow14_TurnLights,Fellow15_TurnLights,Fellow16_TurnLights,Fellow17_TurnLights,Fellow18_TurnLights,Fellow19_TurnLights,Fellow20_TurnLights,Fellow21_TurnLights,Fellow22_TurnLights,Fellow23_TurnLights,Fellow24_TurnLights,Fellow25_TurnLights,Fellow26_TurnLights,Fellow27_TurnLights,Fellow28_TurnLights,Fellow29_TurnLights,Fellow30_TurnLights,Fellow1_DoorFL,Fellow2_DoorFL,Fellow3_DoorFL,Fellow4_DoorFL,Fellow5_DoorFL,Fellow6_DoorFL,Fellow7_DoorFL,Fellow8_DoorFL,Fellow9_DoorFL,Fellow10_DoorFL,Fellow11_DoorFL,Fellow12_DoorFL,Fellow13_DoorFL,Fellow14_DoorFL,Fellow15_DoorFL,Fellow16_DoorFL,Fellow17_DoorFL,Fellow18_DoorFL,Fellow19_DoorFL,Fellow20_DoorFL,Fellow21_DoorFL,Fellow22_DoorFL,Fellow23_DoorFL,Fellow24_DoorFL,Fellow25_DoorFL,Fellow26_DoorFL,Fellow27_DoorFL,Fellow28_DoorFL,Fellow29_DoorFL,Fellow30_DoorFL,Fellow1_DoorFR,Fellow2_DoorFR,Fellow3_DoorFR,Fellow4_DoorFR,Fellow5_DoorFR,Fellow6_DoorFR,Fellow7_DoorFR,Fellow8_DoorFR,Fellow9_DoorFR,Fellow10_DoorFR,Fellow11_DoorFR,Fellow12_DoorFR,Fellow13_DoorFR,Fellow14_DoorFR,Fellow15_DoorFR,Fellow16_DoorFR,Fellow17_DoorFR,Fellow18_DoorFR,Fellow19_DoorFR,Fellow20_DoorFR,Fellow21_DoorFR,Fellow22_DoorFR,Fellow23_DoorFR,Fellow24_DoorFR,Fellow25_DoorFR,Fellow26_DoorFR,Fellow27_DoorFR,Fellow28_DoorFR,Fellow29_DoorFR,Fellow30_DoorFR,Fellow1_DoorRL,Fellow2_DoorRL,Fellow3_DoorRL,Fellow4_DoorRL,Fellow5_DoorRL,Fellow6_DoorRL,Fellow7_DoorRL,Fellow8_DoorRL,Fellow9_DoorRL,Fellow10_DoorRL,Fellow11_DoorRL,Fellow12_DoorRL,Fellow13_DoorRL,Fellow14_DoorRL,Fellow15_DoorRL,Fellow16_DoorRL,Fellow17_DoorRL,Fellow18_DoorRL,Fellow19_DoorRL,Fellow20_DoorRL,Fellow21_DoorRL,Fellow22_DoorRL,Fellow23_DoorRL,Fellow24_DoorRL,Fellow25_DoorRL,Fellow26_DoorRL,Fellow27_DoorRL,Fellow28_DoorRL,Fellow29_DoorRL,Fellow30_DoorRL,Fellow1_DoorRR,Fellow2_DoorRR,Fellow3_DoorRR,Fellow4_DoorRR,Fellow5_DoorRR,Fellow6_DoorRR,Fellow7_DoorRR,Fellow8_DoorRR,Fellow9_DoorRR,Fellow10_DoorRR,Fellow11_DoorRR,Fellow12_DoorRR,Fellow13_DoorRR,Fellow14_DoorRR,Fellow15_DoorRR,Fellow16_DoorRR,Fellow17_DoorRR,Fellow18_DoorRR,Fellow19_DoorRR,Fellow20_DoorRR,Fellow21_DoorRR,Fellow22_DoorRR,Fellow23_DoorRR,Fellow24_DoorRR,Fellow25_DoorRR,Fellow26_DoorRR,Fellow27_DoorRR,Fellow28_DoorRR,Fellow29_DoorRR,Fellow30_DoorRR,Fellow1_Hood,Fellow2_Hood,Fellow3_Hood,Fellow4_Hood,Fellow5_Hood,Fellow6_Hood,Fellow7_Hood,Fellow8_Hood,Fellow9_Hood,Fellow10_Hood,Fellow11_Hood,Fellow12_Hood,Fellow13_Hood,Fellow14_Hood,Fellow15_Hood,Fellow16_Hood,Fellow17_Hood,Fellow18_Hood,Fellow19_Hood,Fellow20_Hood,Fellow21_Hood,Fellow22_Hood,Fellow23_Hood,Fellow24_Hood,Fellow25_Hood,Fellow26_Hood,Fellow27_Hood,Fellow28_Hood,Fellow29_Hood,Fellow30_Hood,Fellow1_Trunk,Fellow2_Trunk,Fellow3_Trunk,Fellow4_Trunk,Fellow5_Trunk,Fellow6_Trunk,Fellow7_Trunk,Fellow8_Trunk,Fellow9_Trunk,Fellow10_Trunk,Fellow11_Trunk,Fellow12_Trunk,Fellow13_Trunk,Fellow14_Trunk,Fellow15_Trunk,Fellow16_Trunk,Fellow17_Trunk,Fellow18_Trunk,Fellow19_Trunk,Fellow20_Trunk,Fellow21_Trunk,Fellow22_Trunk,Fellow23_Trunk,Fellow24_Trunk,Fellow25_Trunk,Fellow26_Trunk,Fellow27_Trunk,Fellow28_Trunk,Fellow29_Trunk,Fellow30_Trunk
  VehicleInitStates : BusSelector  OutputSignals=q_dt_Vehicle_Init[6x1],Enable_v_Init[0|1]
  wires:
  ASMSignalBus/1 -> BusSelector_1/1
  BusSelector_1/1 -> Maneuver/1  "<Maneuver>"
  Maneuver/1 -> ManeuverScheduler/1  "<ManeuverScheduler>"
  ManeuverScheduler/1 -> MdlControl/1  "<MdlControl>"
  ManeuverScheduler/2 -> InitialVehStates/1  "<InitialVehStates>"
  ManeuverScheduler/3 -> ModeSignals/1  "<ModeSignals>"
  ManeuverScheduler/4 -> RefSignals/1  "<RefSignals>"
  ManeuverScheduler/5 -> Parameters/1  "<Parameters>"
  ManeuverScheduler/6 -> UserSignals/1  "<UserSignals>"
  ManeuverScheduler/7 -> Info/1  "<Info>"
  Maneuver/2 -> UserSignals_Customized/1  "<UserSignals_Customized>"
  Maneuver/3 -> VehicleInitStates/1  "<VehicleInitStates>"
  Maneuver/4 -> Testbench/1  "<Testbench>"
  Maneuver/5 -> ParkingBrake/1  "<ParkingBrake>"
  Maneuver/6 -> StartButton/1  "<StartButton>"
  BusSelector_1/2 -> Road/1  "<Road>"
  Road/1 -> Road_Init/1  "<Road_Init>"
  Road/2 -> Road_ASMVeh/1  "<Road_ASMVeh>"
  Road/3 -> Road_ContactPoints/1  "<Road_ContactPoints>"
  Road/4 -> Road_Preview/1  "<Road_Preview>"
  Road/5 -> Road_Info/1  "<Road_Info>"
  Road_Info/4 -> Dist_Response_Maneuver/1  "<Dist_Response_Maneuver>"
  Road_Info/15 -> Trf_Driver_Data/1  "<Trf_Driver_Data>"
  Road_Info/16 -> Line_Sensor_Data/1  "<Line_Sensor_Data>"
  Road/6 -> Road_TrafficFellows/1  "<Road_TrafficFellows>"
  Road_TrafficFellows/18 -> Dist_Response_Traffic/1  "<Dist_Response_Traffic>"
  Road/7 -> UserSignals1/1  "<UserSignals>"
  Road/9 -> UserSignals_Customized1/1  "<UserSignals_Customized>"
  Road/10 -> Pos_Vehicle_GPS[Long;Lat][deg]/1  "<Pos_Vehicle_GPS[Long;Lat][deg]>"
  Road/11 -> Ambient/1  "<Ambient>"
  Road/12 -> LaneSensor_Dynamic/1  "<LaneSensor_Dynamic>"
  LaneSensor_Dynamic/1 -> Parameters1/1  "<Parameters>"
  LaneSensor_Dynamic/2 -> Sensor_Output/1  "<Sensor_Output>"
  Sensor_Output/1 -> SFunction_Info/1  "<SFunction_Info>"
  Sensor_Output/2 -> Network_Item/1  "<Network_Item>"
  Sensor_Output/3 -> CurrentLane/1  "<CurrentLane>"
  CurrentLane/1 -> Common/1  "<Common>"
  CurrentLane/2 -> LeftSide/1  "<LeftSide>"
  CurrentLane/3 -> RightSide/1  "<RightSide>"
  Sensor_Output/4 -> Lanes_Left/1  "<Lanes_Left>"
  Sensor_Output/5 -> Lanes_Right/1  "<Lanes_Right>"
  Sensor_Output/6 -> Measurement_Points/1  "<Measurement_Points>"
  Road/13 -> Lane_Network/1  "<Lane_Network>"
  BusSelector_1/3 -> Traffic/1  "<Traffic>"
  Traffic/1 -> Traffic_Signals_toEnvironment/1  "<Traffic_Signals_toEnvironment>"
  Traffic_Signals_toEnvironment/14 -> Info1/1  "<Info>"
  Traffic_Signals_toEnvironment/20 -> Pos_Fellows_MainPnt_CoorSys_E[x;y;z][m]/1  "<Pos_Fellows_MainPnt_CoorSys_E[x;y;z][m]>"
  Traffic_Signals_toEnvironment/21 -> Angle_Fellows[x;y;z][deg]/1  "<Angle_Fellows[x;y;z][deg]>"
  Traffic_Signals_toEnvironment/25 -> UserSignals_Customized2/1  "<UserSignals_Customized>"
  UserSignals_Customized2/2 -> DriverMonitoring/1  "<DriverMonitoring>"
  Traffic_Signals_toEnvironment/26 -> Control/1  "<Control>"
  Traffic/2 -> FellowSignalLabels/1  "<FellowSignalLabels>"
  Traffic/3 -> ObjectParameters/1  "<ObjectParameters>"
  ObjectParameters/1 -> FellowParameters/1  "<FellowParameters>"
  FellowParameters/1 -> Info2/1  "<Info>"
  ObjectParameters/2 -> TrafficObjects/1  "<TrafficObjects>"
  ObjectParameters/3 -> DiscreteObjects/1  "<DiscreteObjects>"
  BusSelector_1/4 -> GroundTruth/1  "<GroundTruth>"
  GroundTruth/1 -> Control1/1  "<Control>"
  GroundTruth/2 -> Info3/1  "<Info>"
  GroundTruth/3 -> Data/1  "<Data>"
  GroundTruth/4 -> Data_Access/1  "<Data_Access>"
  GroundTruth/5 -> OpenSimulationInterface/1  "<OpenSimulationInterface>"
  BusSelector_1/5 -> Sensors/1  "<Sensors>"
  Sensors/1 -> Collision_Sensor/1  "<Collision_Sensor>"
  Collision_Sensor/1 -> Collision_Sensor_1/1  "<Collision_Sensor_1>"
  Collision_Sensor_1/1 -> Info4/1  "<Info>"
  Collision_Sensor_1/2 -> SensorOutput/1  "<SensorOutput>"
  Sensors/2 -> TrafficSign_Sensor_Dyn/1  "<TrafficSign_Sensor_Dyn>"
  TrafficSign_Sensor_Dyn/1 -> Sensor_Front_1/1  "<Sensor_Front_1>"
  Sensor_Front_1/1 -> Info5/1  "<Info>"
  Sensor_Front_1/2 -> SensorOutput[]/1  "<SensorOutput[]>"
  Sensor_Front_1/3 -> Parameters2/1  "<Parameters>"
  Sensors/3 -> Object_Sensor_3D_1/1  "<Object_Sensor_3D_1>"
  Object_Sensor_3D_1/1 -> Parameter/1  "<Parameter>"
  Object_Sensor_3D_1/2 -> SensorIndex/1  "<SensorIndex>"
  Object_Sensor_3D_1/3 -> Info6/1  "<Info>"
  Object_Sensor_3D_1/4 -> SensorOutput1/1  "<SensorOutput>"
  Object_Sensor_3D_1/5 -> SensorTimeStamp/1  "<SensorTimeStamp>"
  Object_Sensor_3D_1/6 -> RadarEffects/1  "<RadarEffects>"
  Object_Sensor_3D_1/7 -> CustomPoints/1  "<CustomPoints>"
  Object_Sensor_3D_1/8 -> ObjectData/1  "<ObjectData>"
  ObjectData/1 -> Object_Positions/1  "<Object_Positions>"
  ObjectData/2 -> Object_Properties_Box/1  "<Object_Properties_Box>"
  ObjectData/3 -> Object_Custom_Values/1  "<Object_Custom_Values>"
  Sensors/4 -> Object_Sensor_3D_2/1  "<Object_Sensor_3D_2>"
  Object_Sensor_3D_2/1 -> Parameter1/1  "<Parameter>"
  Object_Sensor_3D_2/2 -> SensorIndex1/1  "<SensorIndex>"
  Object_Sensor_3D_2/3 -> Info7/1  "<Info>"
  Object_Sensor_3D_2/4 -> SensorOutput2/1  "<SensorOutput>"
  Object_Sensor_3D_2/5 -> SensorTimeStamp1/1  "<SensorTimeStamp>"
  Object_Sensor_3D_2/6 -> RadarEffects1/1  "<RadarEffects>"
  Object_Sensor_3D_2/7 -> CustomPoints1/1  "<CustomPoints>"
  Object_Sensor_3D_2/8 -> ObjectData1/1  "<ObjectData>"
  ObjectData1/1 -> Object_Positions1/1  "<Object_Positions>"
  ObjectData1/2 -> Object_Properties_Box1/1  "<Object_Properties_Box>"
  ObjectData1/3 -> Object_Custom_Values1/1  "<Object_Custom_Values>"
  Sensors/5 -> Object_Sensor_2D_1/1  "<Object_Sensor_2D_1>"
  Object_Sensor_2D_1/1 -> Parameters3/1  "<Parameters>"
  Object_Sensor_2D_1/2 -> SensorIndex2/1  "<SensorIndex>"
  Object_Sensor_2D_1/3 -> SensorStatus/1  "<SensorStatus>"
  Object_Sensor_2D_1/4 -> SensorOutput3/1  "<SensorOutput>"
  Object_Sensor_2D_1/5 -> Info8/1  "<Info>"
  Object_Sensor_2D_1/6 -> ObjectData2/1  "<ObjectData>"
  ObjectData2/1 -> Object_Positions2/1  "<Object_Positions>"
  ObjectData2/2 -> Object_Properties_Box2/1  "<Object_Properties_Box>"
  ObjectData2/3 -> Object_Custom_Values2/1  "<Object_Custom_Values>"
  ContentID/1 -> Terminator/1
  MdlControl/1 -> SignalFilter/1  "<Reset_VehicleStates[0|1]>"
  MdlControl/2 -> SignalFilter/2  "<RoadControl[]>"
  MdlControl/3 -> SignalFilter/3  "<Get_VehPos_Trigger[]>"
  MdlControl/4 -> SignalFilter/4  "<Keep_VehiclePosition[0|1]>"
  InitialVehStates/1 -> SignalFilter/5  "<s_Vehicle_Init[m]>"
  InitialVehStates/2 -> SignalFilter/6  "<d_Vehicle_Init[m]>"
  InitialVehStates/3 -> SignalFilter/7  "<LaneIdx_Vehicle_Init[]>"
  InitialVehStates/4 -> SignalFilter/8  "<Pos_z_Vehicle_Rel_Init[m]>"
  InitialVehStates/5 -> SignalFilter/9  "<Angle_Yaw_Vehicle_Rel_Init[deg]>"
  InitialVehStates/6 -> SignalFilter/10  "<v_Vehicle_Init[km|h]>"
  InitialVehStates/7 -> SignalFilter/11  "<Route_Id_Init[]>"
  InitialVehStates/8 -> SignalFilter/12  "<Route_Direction_Init[]>"
  ModeSignals/1 -> SignalFilter/13  "<Mode_AccBr[1Stim|2Driver]>"
  ModeSignals/2 -> SignalFilter/14  "<Mode_GearClutch[1Stim|2Driver|3OpenClutch|4RefGear]>"
  ModeSignals/3 -> SignalFilter/15  "<Mode_Steer[1Stim|2Driver|3Fix]>"
  ModeSignals/4 -> SignalFilter/16  "<Mode_Road[1NoRoad|2Straight|3Circle|4Road]>"
  ModeSignals/5 -> SignalFilter/17  "<LatDriver[1LatCtrl1|2LatCtrl2]>"
  ModeSignals/6 -> SignalFilter/18  "<Mode_LatCtrl[1Pos|2Yaw]>"
  ModeSignals/7 -> SignalFilter/19  "<Mode_AdaptVelocityToRoad[1Off|2On]>"
  ModeSignals/8 -> SignalFilter/20  "<Mode_ForceToRoad[1Off|2On]>"
  ModeSignals/9 -> SignalFilter/21  "<Mode_SelectorLever[1Stim|2Driver]>"
  ModeSignals/10 -> SignalFilter/22  "<Mode_CurvatureCalculation[1Road|2Driver]>"
  ModeSignals/11 -> SignalFilter/23  "<Mode_TrafficDriver[1Off|2On]>"
  ModeSignals/12 -> SignalFilter/24  "<Mode_RelativeLane[0CenterLane|1PreferredLane]>"
  RefSignals/1 -> SignalFilter/25  "<Pos_AccPedal_Maneuver[%]>"
  RefSignals/2 -> SignalFilter/26  "<Pos_BrakePedal_Maneuver[%]>"
  RefSignals/3 -> SignalFilter/27  "<Pos_ClutchPedal_Maneuver[%]>"
  RefSignals/4 -> SignalFilter/28  "<Gear_Maneuver[]>"
  RefSignals/5 -> SignalFilter/29  "<Angle_SteeringWheel_Maneuver[deg]>"
  RefSignals/6 -> SignalFilter/30  "<v_Vehicle_Ref_Maneuver[m|s]>"
  RefSignals/7 -> SignalFilter/31  "<v_Vehicle_Ref_Maneuver[km|h]>"
  RefSignals/8 -> SignalFilter/32  "<d_Maneuver[m]>"
  RefSignals/9 -> SignalFilter/33  "<LaneIdx_Maneuver[]>"
  RefSignals/10 -> Reshape_34/1  "<Dist_Def_Maneuver[]>"
  Reshape_34/1 -> SignalFilter/34
  RefSignals/11 -> SignalFilter/35  "<v_Vehicle_Ref_Preview_Maneuver[m|s]>"
  RefSignals/12 -> SignalFilter/36  "<v_Vehicle_Ref_Preview_State[0Invalid|1CurrentSeg|2NextSeg]>"
  RefSignals/13 -> SignalFilter/37  "<Sw_SteeringMode_Maneuver[1Angle|2Trq]>"
  RefSignals/14 -> SignalFilter/38  "<Trq_Steering_Maneuver[Nm]>"
  RefSignals/15 -> SignalFilter/39  "<SelectorLever_Maneuver[]>"
  RefSignals/16 -> Reshape_40/1  "<Dist_Def_Refline_Maneuver[]>"
  Reshape_40/1 -> SignalFilter/40
  Parameters/1 -> SignalFilter/41  "<a_x_Max[m|s2]>"
  Parameters/2 -> SignalFilter/42  "<a_x_Brake_Threshold[m|s2]>"
  Parameters/3 -> SignalFilter/43  "<a_y_Max[m|s2]>"
  Parameters/4 -> SignalFilter/44  "<Curv_Road_Circle[1|m]>"
  Parameters/5 -> SignalFilter/45  "<Gear_Max[]>"
  Parameters/6 -> SignalFilter/46  "<Width_Deadzone_LatCtrl[m]>"
  Parameters/7 -> SignalFilter/47  "<v_Lat[m|s]>"
  Parameters/8 -> SignalFilter/48  "<Object_Type_ID[]>"
  Parameters/9 -> SignalFilter/49  "<Driver_Type_Index[]>"
  UserSignals/1 -> SignalFilter/50  "<User1[]>"
  UserSignals/2 -> SignalFilter/51  "<User2[]>"
  UserSignals/3 -> SignalFilter/52  "<User3[]>"
  UserSignals/4 -> SignalFilter/53  "<User4[]>"
  UserSignals/5 -> SignalFilter/54  "<User5[]>"
  UserSignals/6 -> SignalFilter/55  "<User6[]>"
  UserSignals/7 -> SignalFilter/56  "<User7[]>"
  UserSignals/8 -> SignalFilter/57  "<User8[]>"
  UserSignals/9 -> SignalFilter/58  "<User9[]>"
  UserSignals/10 -> SignalFilter/59  "<User10[]>"
  UserSignals/11 -> SignalFilter/60  "<User11[]>"
  UserSignals/12 -> SignalFilter/61  "<User12[]>"
  UserSignals/13 -> SignalFilter/62  "<User13[]>"
  UserSignals/14 -> SignalFilter/63  "<User14[]>"
  UserSignals/15 -> SignalFilter/64  "<User15[]>"
  UserSignals/16 -> SignalFilter/65  "<User16[]>"
  UserSignals/17 -> SignalFilter/66  "<User17[]>"
  UserSignals/18 -> SignalFilter/67  "<User18[]>"
  UserSignals/19 -> SignalFilter/68  "<User19[]>"
  UserSignals/20 -> SignalFilter/69  "<User20[]>"
  UserSignals/21 -> SignalFilter/70  "<User21[]>"
  UserSignals/22 -> SignalFilter/71  "<User22[]>"
  UserSignals/23 -> SignalFilter/72  "<User23[]>"
  UserSignals/24 -> SignalFilter/73  "<User24[]>"
  UserSignals/25 -> SignalFilter/74  "<User25[]>"
  UserSignals/26 -> SignalFilter/75  "<User26[]>"
  UserSignals/27 -> SignalFilter/76  "<User27[]>"
  UserSignals/28 -> SignalFilter/77  "<User28[]>"
  UserSignals/29 -> SignalFilter/78  "<User29[]>"
  UserSignals/30 -> SignalFilter/79  "<User30[]>"
  Info/1 -> SignalFilter/80  "<CurrentSegment[]>"
  Info/2 -> SignalFilter/81  "<t_local[s]>"
  Info/3 -> SignalFilter/82  "<s_local[m]>"
  Info/4 -> SignalFilter/83  "<ManeuverTime[s]>"
  Info/5 -> SignalFilter/84  "<ManeuverState[]>"
  Info/6 -> SignalFilter/85  "<ErrorFlag[]>"
  Info/7 -> SignalFilter/86  "<CurrentSequence[]>"
  UserSignals_Customized/1 -> SignalFilter/87  "<ExternalSegmentEnd_Mode[]>"
  UserSignals_Customized/2 -> SignalFilter/88  "<ExternalSegmentEnd_Value[]>"
  UserSignals_Customized/3 -> SignalFilter/89  "<ASM_Vehicle_TurnLights[]>"
  UserSignals_Customized/4 -> SignalFilter/90  "<ECU_Commands[]>"
  UserSignals_Customized/5 -> SignalFilter/91  "<Mnv_DataStream_5[]>"
  UserSignals_Customized/6 -> SignalFilter/92  "<Mnv_DataStream_6[]>"
  UserSignals_Customized/7 -> SignalFilter/93  "<Mnv_DataStream_7[]>"
  UserSignals_Customized/8 -> SignalFilter/94  "<Mnv_DataStream_8[]>"
  UserSignals_Customized/9 -> SignalFilter/95  "<Mnv_DoorFL[]>"
  UserSignals_Customized/10 -> SignalFilter/96  "<Mnv_DoorFR[]>"
  UserSignals_Customized/11 -> SignalFilter/97  "<Mnv_DoorRL[]>"
  UserSignals_Customized/12 -> SignalFilter/98  "<Mnv_DoorRR[]>"
  UserSignals_Customized/13 -> SignalFilter/99  "<Mnv_Hood[]>"
  UserSignals_Customized/14 -> SignalFilter/100  "<Mnv_Trunk[]>"
  VehicleInitStates/1 -> Reshape_101/1  "<q_dt_Vehicle_Init[6x1]>"
  Reshape_101/1 -> SignalFilter/101
  VehicleInitStates/2 -> DataTypeConversion_102/1  "<Enable_v_Init[0|1]>"
  DataTypeConversion_102/1 -> SignalFilter/102
  Testbench/1 -> SignalFilter/103  "<Sw_Testbench[0Off|1On]>"
  Testbench/2 -> SignalFilter/104  "<EngOpNum[]>"
  Testbench/3 -> SignalFilter/105  "<n_Engine_Set[rpm]>"
  ParkingBrake/1 -> SignalFilter/106  "<Sw_ParkingBrake[0Off|1On]>"
  StartButton/1 -> SignalFilter/107  "<Sw_StartButton[0Off|1On]>"
  StartButton/2 -> SignalFilter/108  "<Mode_StartButtonState[1Stim|2SoftECU]>"
  StartButton/3 -> SignalFilter/109  "<State_StartButton[-1PowerOff|0Acc|1PowerOn|2StarterOn]>"
  Maneuver/7 -> SignalFilter/110  "<Sw_TipShift[-1Down|0Off|1Up]>"
  Road_Init/1 -> Reshape_111/1  "<Pos_Vehicle_Init_CoorSys_E[x;y;z][m]>"
  Reshape_111/1 -> SignalFilter/111
  Road_Init/2 -> Reshape_112/1  "<Angle_Vehicle_Init_CoorSys_E[x;y;z][rad]>"
  Reshape_112/1 -> SignalFilter/112
  Road_ASMVeh/1 -> SignalFilter/113  "<s_Veh_Road[m]>"
  Road_ASMVeh/2 -> SignalFilter/114  "<s_Total_Veh_Road[m]>"
  Road_ASMVeh/3 -> SignalFilter/115  "<d_Total_Veh_Road[m]>"
  Road_ASMVeh/4 -> SignalFilter/116  "<s_Veh_Road_Trj[m]>"
  Road_ASMVeh/5 -> SignalFilter/117  "<LaneIdx_Total_Veh_Road[]>"
  Road_ASMVeh/6 -> SignalFilter/118  "<Curv_Veh_Road[1|m]>"
  Road_ASMVeh/7 -> SignalFilter/119  "<Pos_x_Ref_Veh_Road[m]>"
  Road_ASMVeh/8 -> SignalFilter/120  "<Pos_y_Ref_Veh_Road[m]>"
  Road_ASMVeh/9 -> SignalFilter/121  "<Angle_Yaw_Veh_Road[deg]>"
  Road_ASMVeh/10 -> SignalFilter/122  "<Slope_Veh_Road[%]>"
  Road_ASMVeh/11 -> Reshape_123/1  "<v_Wind_Coor_Sys_E[x;y;z][m|s]>"
  Reshape_123/1 -> SignalFilter/123
  Road_ASMVeh/12 -> SignalFilter/124  "<Slope_Lateral_Veh_Road[deg]>"
  Road_ContactPoints/1 -> Reshape_125/1  "<Pos_z_CP[:][m]>"
  Reshape_125/1 -> SignalFilter/125
  Road_ContactPoints/2 -> Reshape_126/1  "<Fric_Coeff_CP[:][]>"
  Reshape_126/1 -> SignalFilter/126
  Road_ContactPoints/3 -> Reshape_127/1  "<UnitVec_z_CP[:][x;y;z]>"
  Reshape_127/1 -> SignalFilter/127
  Road_ContactPoints/4 -> Reshape_128/1  "<Sw_Tire_Parameter_Set_CP[:][1|2|3|4]>"
  Reshape_128/1 -> SignalFilter/128
  Road_Preview/1 -> Reshape_129/1  "<Pos_x_Preview_Road[m]>"
  Reshape_129/1 -> SignalFilter/129
  Road_Preview/2 -> Reshape_130/1  "<Pos_y_Preview_Road[m]>"
  Reshape_130/1 -> SignalFilter/130
  Road_Preview/3 -> Reshape_131/1  "<Curv_Preview_Road[1|m]>"
  Reshape_131/1 -> SignalFilter/131
  Road_Preview/4 -> Reshape_132/1  "<Speed_Limit_Preview_Road[km|h]>"
  Reshape_132/1 -> SignalFilter/132
  Road_Preview/5 -> Reshape_133/1  "<Pos_z_Preview_Road[m]>"
  Reshape_133/1 -> SignalFilter/133
  Road_Preview/6 -> Reshape_134/1  "<Roll_Preview_Road[deg]>"
  Reshape_134/1 -> SignalFilter/134
  Road_Preview/7 -> Reshape_135/1  "<Pitch_Preview_Road[deg]>"
  Reshape_135/1 -> SignalFilter/135
  Road_Preview/8 -> Reshape_136/1  "<x_Preview_DriverCurv[m]>"
  Reshape_136/1 -> SignalFilter/136
  Road_Preview/9 -> Reshape_137/1  "<y_Preview_DriverCurv[m]>"
  Reshape_137/1 -> SignalFilter/137
  Road_Info/1 -> SignalFilter/138  "<RoadState[]>"
  Road_Info/2 -> SignalFilter/139  "<RouteLength_Veh[m]>"
  Road_Info/3 -> SignalFilter/140  "<Flag_RouteClosed_Veh[0|1]>"
  Dist_Response_Maneuver/1 -> SignalFilter/141  "<Distance_xy[m]>"
  Dist_Response_Maneuver/2 -> SignalFilter/142  "<Distance_z[m]>"
  Road_Info/5 -> SignalFilter/143  "<Speed_Limit_Veh[km|h]>"
  Road_Info/6 -> SignalFilter/144  "<Network_Item_Type_Veh[]>"
  Road_Info/7 -> SignalFilter/145  "<Network_Item_Id_Veh[]>"
  Road_Info/8 -> SignalFilter/146  "<RoadSegment_Veh[]>"
  Road_Info/9 -> SignalFilter/147  "<LaneSection_Veh[]>"
  Road_Info/10 -> SignalFilter/148  "<RoadWidth_Veh[m]>"
  Road_Info/11 -> SignalFilter/149  "<Network_Load_Idx[]>"
  Road_Info/12 -> SignalFilter/150  "<d_Veh_Ref_Line[m]>"
  Road_Info/13 -> SignalFilter/151  "<Dist_Border_Left[m]>"
  Road_Info/14 -> SignalFilter/152  "<Dist_Border_Right[m]>"
  Trf_Driver_Data/1 -> SignalFilter/153  "<Route_Idx_Veh[]>"
  Trf_Driver_Data/2 -> Reshape_154/1  "<Route_Idx_Fellows[]>"
  Reshape_154/1 -> SignalFilter/154
  Trf_Driver_Data/3 -> Reshape_155/1  "<RoadNetworkData>"
  Reshape_155/1 -> DataTypeConversion_155/1
  DataTypeConversion_155/1 -> SignalFilter/155
  Line_Sensor_Data/1 -> Reshape_156/1  "<RoadNetworkData>"
  Reshape_156/1 -> DataTypeConversion_156/1
  DataTypeConversion_156/1 -> SignalFilter/156
  Road_Info/17 -> Reshape_157/1  "<V2X_Data[]>"
  Reshape_157/1 -> DataTypeConversion_157/1
  DataTypeConversion_157/1 -> SignalFilter/157
  Road_TrafficFellows/1 -> Reshape_158/1  "<Pos_x_Fellows_Road[m]>"
  Reshape_158/1 -> SignalFilter/158
  Road_TrafficFellows/2 -> Reshape_159/1  "<Pos_y_Fellows_Road[m]>"
  Reshape_159/1 -> SignalFilter/159
  Road_TrafficFellows/3 -> Reshape_160/1  "<Pos_z_Fellows_Road[m]>"
  Reshape_160/1 -> SignalFilter/160
  Road_TrafficFellows/4 -> Reshape_161/1  "<Angle_Yaw_Fellows_Road[deg]>"
  Reshape_161/1 -> SignalFilter/161
  Road_TrafficFellows/5 -> Reshape_162/1  "<Angle_Pitch_Fellows_Road[deg]>"
  Reshape_162/1 -> SignalFilter/162
  Road_TrafficFellows/6 -> Reshape_163/1  "<Angle_Roll_Fellows_Road[deg]>"
  Reshape_163/1 -> SignalFilter/163
  Road_TrafficFellows/7 -> Reshape_164/1  "<Curv_Fellows_Road[1|m]>"
  Reshape_164/1 -> SignalFilter/164
  Road_TrafficFellows/8 -> Reshape_165/1  "<d_Total_Fellows_Road[m]>"
  Reshape_165/1 -> SignalFilter/165
  Road_TrafficFellows/9 -> Reshape_166/1  "<LaneIdx_Total_Fellows_Road[]>"
  Reshape_166/1 -> SignalFilter/166
  Road_TrafficFellows/10 -> Reshape_167/1  "<RoadSegment_Fellows[]>"
  Reshape_167/1 -> SignalFilter/167
  Road_TrafficFellows/11 -> Reshape_168/1  "<LaneSection_Fellows[]>"
  Reshape_168/1 -> SignalFilter/168
  Road_TrafficFellows/12 -> Reshape_169/1  "<Speed_Limit_Fellows[]>"
  Reshape_169/1 -> SignalFilter/169
  Road_TrafficFellows/13 -> Reshape_170/1  "<Network_Item_Type_Fellows[]>"
  Reshape_170/1 -> SignalFilter/170
  Road_TrafficFellows/14 -> Reshape_171/1  "<Network_Item_Id_Fellows[]>"
  Reshape_171/1 -> SignalFilter/171
  Road_TrafficFellows/15 -> Reshape_172/1  "<d_Fellows_RefLine[m]>"
  Reshape_172/1 -> SignalFilter/172
  Road_TrafficFellows/16 -> Reshape_173/1  "<RouteLength_Fellows[m]>"
  Reshape_173/1 -> SignalFilter/173
  Road_TrafficFellows/17 -> Reshape_174/1  "<Flag_RouteClosed_Fellows[0|1]>"
  Reshape_174/1 -> SignalFilter/174
  Dist_Response_Traffic/1 -> Reshape_175/1  "<Distance_xy[m]>"
  Reshape_175/1 -> SignalFilter/175
  Dist_Response_Traffic/2 -> Reshape_176/1  "<Distance_z[m]>"
  Reshape_176/1 -> SignalFilter/176
  Road_TrafficFellows/19 -> Reshape_177/1  "<Angle_Yaw_Fellows_RoadRefline[deg]>"
  Reshape_177/1 -> SignalFilter/177
  UserSignals1/1 -> SignalFilter/178  "<User1[]>"
  UserSignals1/2 -> SignalFilter/179  "<User2[]>"
  UserSignals1/3 -> SignalFilter/180  "<User3[]>"
  UserSignals1/4 -> SignalFilter/181  "<User4[]>"
  UserSignals1/5 -> SignalFilter/182  "<User5[]>"
  UserSignals1/6 -> SignalFilter/183  "<User6[]>"
  UserSignals1/7 -> SignalFilter/184  "<User7[]>"
  UserSignals1/8 -> SignalFilter/185  "<User8[]>"
  UserSignals1/9 -> SignalFilter/186  "<User9[]>"
  UserSignals1/10 -> SignalFilter/187  "<User10[]>"
  Road/8 -> Reshape_188/1  "<TrafficObject_Data[]>"
  Reshape_188/1 -> DataTypeConversion_188/1
  DataTypeConversion_188/1 -> SignalFilter/188
  UserSignals_Customized1/1 -> SignalFilter/189  "<GPS_Method[]>"
  UserSignals_Customized1/2 -> SignalFilter/190  "<Const_Offset_Lat[deg]>"
  UserSignals_Customized1/3 -> SignalFilter/191  "<Const_Offset_Long[deg]>"
  UserSignals_Customized1/4 -> SignalFilter/192  "<User4[]>"
  UserSignals_Customized1/5 -> SignalFilter/193  "<User5[]>"
  UserSignals_Customized1/6 -> SignalFilter/194  "<User6[]>"
  UserSignals_Customized1/7 -> SignalFilter/195  "<User7[]>"
  UserSignals_Customized1/8 -> SignalFilter/196  "<User8[]>"
  UserSignals_Customized1/9 -> SignalFilter/197  "<User9[]>"
  UserSignals_Customized1/10 -> SignalFilter/198  "<User10[]>"
  Pos_Vehicle_GPS[Long;Lat][deg]/1 -> SignalFilter/199  "<Longitude[deg]>"
  Pos_Vehicle_GPS[Long;Lat][deg]/2 -> SignalFilter/200  "<Latitude[deg]>"
  Pos_Vehicle_GPS[Long;Lat][deg]/3 -> SignalFilter/201  "<Heading[deg]>"
  Ambient/1 -> SignalFilter/202  "<T_Ambient[degC]>"
  Ambient/2 -> SignalFilter/203  "<p_Ambient[Pa]>"
  Parameters1/1 -> Reshape_204/1  "<Enable_Evaluation[0|1]>"
  Reshape_204/1 -> SignalFilter/204
  Parameters1/2 -> Reshape_205/1  "<Evaluation_Distance[m]>"
  Reshape_205/1 -> SignalFilter/205
  Parameters1/3 -> SignalFilter/206  "<Border_Mode[0Center|1Inner|2Outer]>"
  Parameters1/4 -> SignalFilter/207  "<Enable_Junction_Evaluation[0|1]>"
  Parameters1/5 -> Reshape_208/1  "<Num_Lanes[Left;Right]>"
  Reshape_208/1 -> SignalFilter/208
  Parameters1/6 -> Reshape_209/1  "<Enable_MeasPoint[0|1]>"
  Reshape_209/1 -> SignalFilter/209
  Parameters1/7 -> Reshape_210/1  "<MeasPoint_1_CoorSysV[x;y][m]>"
  Reshape_210/1 -> SignalFilter/210
  Parameters1/8 -> Reshape_211/1  "<MeasPoint_2_CoorSysV[x;y][m]>"
  Reshape_211/1 -> SignalFilter/211
  Parameters1/9 -> Reshape_212/1  "<MeasPoint_3_CoorSysV[x;y][m]>"
  Reshape_212/1 -> SignalFilter/212
  Parameters1/10 -> Reshape_213/1  "<MeasPoint_4_CoorSysV[x;y][m]>"
  Reshape_213/1 -> SignalFilter/213
  Parameters1/11 -> Reshape_214/1  "<MeasPoint_1_CoorSysE[x;y][m]>"
  Reshape_214/1 -> SignalFilter/214
  Parameters1/12 -> Reshape_215/1  "<MeasPoint_2_CoorSysE[x;y][m]>"
  Reshape_215/1 -> SignalFilter/215
  Parameters1/13 -> Reshape_216/1  "<MeasPoint_3_CoorSysE[x;y][m]>"
  Reshape_216/1 -> SignalFilter/216
  Parameters1/14 -> Reshape_217/1  "<MeasPoint_4_CoorSysE[x;y][m]>"
  Reshape_217/1 -> SignalFilter/217
  SFunction_Info/1 -> SignalFilter/218  "<Sfcn_State[0|1]>"
  SFunction_Info/2 -> SignalFilter/219  "<Input_Data_Valid[0|1]>"
  SFunction_Info/3 -> DataTypeConversion_220/1  "<Data_Valid[0|1]>"
  DataTypeConversion_220/1 -> SignalFilter/220
  Network_Item/1 -> Reshape_221/1  "<Network_Item_ID[]>"
  Reshape_221/1 -> SignalFilter/221
  Network_Item/2 -> Reshape_222/1  "<Network_Item_Type[]>"
  Reshape_222/1 -> SignalFilter/222
  Network_Item/3 -> Reshape_223/1  "<Network_Item_Type_Absolute[]>"
  Reshape_223/1 -> SignalFilter/223
  Network_Item/4 -> Reshape_224/1  "<Preferred_Lane_Direct[]>"
  Reshape_224/1 -> SignalFilter/224
  Network_Item/5 -> Reshape_225/1  "<Preferred_Lane_Oncoming[]>"
  Reshape_225/1 -> SignalFilter/225
  Common/1 -> Reshape_226/1  "<LaneID_PrefLane[]>"
  Reshape_226/1 -> SignalFilter/226
  Common/2 -> Reshape_227/1  "<LaneID_Absolute[]>"
  Reshape_227/1 -> SignalFilter/227
  Common/3 -> Reshape_228/1  "<LaneDirection_Absolute[]>"
  Reshape_228/1 -> SignalFilter/228
  Common/4 -> Reshape_229/1  "<LaneDirection_Relative[]>"
  Reshape_229/1 -> SignalFilter/229
  Common/5 -> Reshape_230/1  "<LaneWidth[m]>"
  Reshape_230/1 -> SignalFilter/230
  Common/6 -> Reshape_231/1  "<LaneCurvature[1|m]>"
  Reshape_231/1 -> SignalFilter/231
  Common/7 -> Reshape_232/1  "<Curvature[1|m]>"
  Reshape_232/1 -> SignalFilter/232
  LeftSide/1 -> Reshape_233/1  "<Pos_Left[x;y;z][m]>"
  Reshape_233/1 -> SignalFilter/233
  LeftSide/2 -> Reshape_234/1  "<Yaw_Angle_Left[deg]>"
  Reshape_234/1 -> SignalFilter/234
  LeftSide/3 -> Reshape_235/1  "<Yaw_Angle_RelVehicle_Left[deg]>"
  Reshape_235/1 -> SignalFilter/235
  LeftSide/4 -> Reshape_236/1  "<Curvature_Left[1|m]>"
  Reshape_236/1 -> SignalFilter/236
  LeftSide/5 -> Reshape_237/1  "<MarkerType_Left[]>"
  Reshape_237/1 -> SignalFilter/237
  LeftSide/6 -> Reshape_238/1  "<MarkerWidth_Left[m]>"
  Reshape_238/1 -> SignalFilter/238
  LeftSide/7 -> Reshape_239/1  "<MarkerColor_Left[]>"
  Reshape_239/1 -> SignalFilter/239
  LeftSide/8 -> Reshape_240/1  "<LineID_1_Left[]>"
  Reshape_240/1 -> SignalFilter/240
  LeftSide/9 -> Reshape_241/1  "<LineID_2_Left[]>"
  Reshape_241/1 -> SignalFilter/241
  LeftSide/10 -> Reshape_242/1  "<Distance_Marker_Left[m]>"
  Reshape_242/1 -> SignalFilter/242
  RightSide/1 -> Reshape_243/1  "<Pos_Right[x;y;z][m]>"
  Reshape_243/1 -> SignalFilter/243
  RightSide/2 -> Reshape_244/1  "<Yaw_Angle_Right[deg]>"
  Reshape_244/1 -> SignalFilter/244
  RightSide/3 -> Reshape_245/1  "<Yaw_Angle_RelVehicle_Right[deg]>"
  Reshape_245/1 -> SignalFilter/245
  RightSide/4 -> Reshape_246/1  "<Curvature_Right[1|m]>"
  Reshape_246/1 -> SignalFilter/246
  RightSide/5 -> Reshape_247/1  "<MarkerType_Right[]>"
  Reshape_247/1 -> SignalFilter/247
  RightSide/6 -> Reshape_248/1  "<MarkerWidth_Right[m]>"
  Reshape_248/1 -> SignalFilter/248
  RightSide/7 -> Reshape_249/1  "<MarkerColor_Right[]>"
  Reshape_249/1 -> SignalFilter/249
  RightSide/8 -> Reshape_250/1  "<LineID_1_Right[]>"
  Reshape_250/1 -> SignalFilter/250
  RightSide/9 -> Reshape_251/1  "<LineID_2_Right[]>"
  Reshape_251/1 -> SignalFilter/251
  RightSide/10 -> Reshape_252/1  "<Distance_Marker_Right[m]>"
  Reshape_252/1 -> SignalFilter/252
  Lanes_Left/1 -> Reshape_253/1  "<LaneID_PrefLane[]>"
  Reshape_253/1 -> SignalFilter/253
  Lanes_Left/2 -> Reshape_254/1  "<LaneID_Absolute[]>"
  Reshape_254/1 -> SignalFilter/254
  Lanes_Left/3 -> Reshape_255/1  "<LaneDirection_Absolute[]>"
  Reshape_255/1 -> SignalFilter/255
  Lanes_Left/4 -> Reshape_256/1  "<LaneDirection_Relative[]>"
  Reshape_256/1 -> SignalFilter/256
  Lanes_Left/5 -> Reshape_257/1  "<LaneWidth[m]>"
  Reshape_257/1 -> SignalFilter/257
  Lanes_Left/6 -> Reshape_258/1  "<LaneCurvature[1|m]>"
  Reshape_258/1 -> SignalFilter/258
  Lanes_Left/7 -> Reshape_259/1  "<Pos_Left[x;y;z][m]>"
  Reshape_259/1 -> SignalFilter/259
  Lanes_Left/8 -> Reshape_260/1  "<Yaw_Angle_Left[deg]>"
  Reshape_260/1 -> SignalFilter/260
  Lanes_Left/9 -> Reshape_261/1  "<Yaw_Angle_RelVehicle_Left[deg]>"
  Reshape_261/1 -> SignalFilter/261
  Lanes_Left/10 -> Reshape_262/1  "<Curvature_Left[1|m]>"
  Reshape_262/1 -> SignalFilter/262
  Lanes_Left/11 -> Reshape_263/1  "<MarkerType_Left[]>"
  Reshape_263/1 -> SignalFilter/263
  Lanes_Left/12 -> Reshape_264/1  "<MarkerWidth_Left[m]>"
  Reshape_264/1 -> SignalFilter/264
  Lanes_Left/13 -> Reshape_265/1  "<MarkerColor_Left[]>"
  Reshape_265/1 -> SignalFilter/265
  Lanes_Left/14 -> Reshape_266/1  "<LineID_1_Left[]>"
  Reshape_266/1 -> SignalFilter/266
  Lanes_Left/15 -> Reshape_267/1  "<LineID_2_Left[]>"
  Reshape_267/1 -> SignalFilter/267
  Lanes_Left/16 -> Reshape_268/1  "<Distance_Marker_Left[m]>"
  Reshape_268/1 -> SignalFilter/268
  Lanes_Left/17 -> Reshape_269/1  "<Pos_Right[x;y;z][m]>"
  Reshape_269/1 -> SignalFilter/269
  Lanes_Left/18 -> Reshape_270/1  "<Yaw_Angle_Right[deg]>"
  Reshape_270/1 -> SignalFilter/270
  Lanes_Left/19 -> Reshape_271/1  "<Yaw_Angle_RelVehicle_Right[deg]>"
  Reshape_271/1 -> SignalFilter/271
  Lanes_Left/20 -> Reshape_272/1  "<Curvature_Right[1|m]>"
  Reshape_272/1 -> SignalFilter/272
  Lanes_Left/21 -> Reshape_273/1  "<MarkerType_Right[]>"
  Reshape_273/1 -> SignalFilter/273
  Lanes_Left/22 -> Reshape_274/1  "<MarkerWidth_Right[m]>"
  Reshape_274/1 -> SignalFilter/274
  Lanes_Left/23 -> Reshape_275/1  "<MarkerColor_Right[]>"
  Reshape_275/1 -> SignalFilter/275
  Lanes_Left/24 -> Reshape_276/1  "<LineID_1_Right[]>"
  Reshape_276/1 -> SignalFilter/276
  Lanes_Left/25 -> Reshape_277/1  "<LineID_2_Right[]>"
  Reshape_277/1 -> SignalFilter/277
  Lanes_Left/26 -> Reshape_278/1  "<Distance_Marker_Right[m]>"
  Reshape_278/1 -> SignalFilter/278
  Lanes_Right/1 -> Reshape_279/1  "<LaneID_PrefLane[]>"
  Reshape_279/1 -> SignalFilter/279
  Lanes_Right/2 -> Reshape_280/1  "<LaneID_Absolute[]>"
  Reshape_280/1 -> SignalFilter/280
  Lanes_Right/3 -> Reshape_281/1  "<LaneDirection_Absolute[]>"
  Reshape_281/1 -> SignalFilter/281
  Lanes_Right/4 -> Reshape_282/1  "<LaneDirection_Relative[]>"
  Reshape_282/1 -> SignalFilter/282
  Lanes_Right/5 -> Reshape_283/1  "<LaneWidth[m]>"
  Reshape_283/1 -> SignalFilter/283
  Lanes_Right/6 -> Reshape_284/1  "<LaneCurvature[1|m]>"
  Reshape_284/1 -> SignalFilter/284
  Lanes_Right/7 -> Reshape_285/1  "<Pos_Left[x;y;z][m]>"
  Reshape_285/1 -> SignalFilter/285
  Lanes_Right/8 -> Reshape_286/1  "<Yaw_Angle_Left[deg]>"
  Reshape_286/1 -> SignalFilter/286
  Lanes_Right/9 -> Reshape_287/1  "<Yaw_Angle_RelVehicle_Left[deg]>"
  Reshape_287/1 -> SignalFilter/287
  Lanes_Right/10 -> Reshape_288/1  "<Curvature_Left[1|m]>"
  Reshape_288/1 -> SignalFilter/288
  Lanes_Right/11 -> Reshape_289/1  "<MarkerType_Left[]>"
  Reshape_289/1 -> SignalFilter/289
  Lanes_Right/12 -> Reshape_290/1  "<MarkerWidth_Left[m]>"
  Reshape_290/1 -> SignalFilter/290
  Lanes_Right/13 -> Reshape_291/1  "<MarkerColor_Left[]>"
  Reshape_291/1 -> SignalFilter/291
  Lanes_Right/14 -> Reshape_292/1  "<LineID_1_Left[]>"
  Reshape_292/1 -> SignalFilter/292
  Lanes_Right/15 -> Reshape_293/1  "<LineID_2_Left[]>"
  Reshape_293/1 -> SignalFilter/293
  Lanes_Right/16 -> Reshape_294/1  "<Distance_Marker_Left[m]>"
  Reshape_294/1 -> SignalFilter/294
  Lanes_Right/17 -> Reshape_295/1  "<Pos_Right[x;y;z][m]>"
  Reshape_295/1 -> SignalFilter/295
  Lanes_Right/18 -> Reshape_296/1  "<Yaw_Angle_Right[deg]>"
  Reshape_296/1 -> SignalFilter/296
  Lanes_Right/19 -> Reshape_297/1  "<Yaw_Angle_RelVehicle_Right[deg]>"
  Reshape_297/1 -> SignalFilter/297
  Lanes_Right/20 -> Reshape_298/1  "<Curvature_Right[1|m]>"
  Reshape_298/1 -> SignalFilter/298
  Lanes_Right/21 -> Reshape_299/1  "<MarkerType_Right[]>"
  Reshape_299/1 -> SignalFilter/299
  Lanes_Right/22 -> Reshape_300/1  "<MarkerWidth_Right[m]>"
  Reshape_300/1 -> SignalFilter/300
  Lanes_Right/23 -> Reshape_301/1  "<MarkerColor_Right[]>"
  Reshape_301/1 -> SignalFilter/301
  Lanes_Right/24 -> Reshape_302/1  "<LineID_1_Right[]>"
  Reshape_302/1 -> SignalFilter/302
  Lanes_Right/25 -> Reshape_303/1  "<LineID_2_Right[]>"
  Reshape_303/1 -> SignalFilter/303
  Lanes_Right/26 -> Reshape_304/1  "<Distance_Marker_Right[m]>"
  Reshape_304/1 -> SignalFilter/304
  Measurement_Points/1 -> Reshape_305/1  "<Distance_MeasPnt_Marker_Left[m]>"
  Reshape_305/1 -> SignalFilter/305
  Measurement_Points/2 -> Reshape_306/1  "<Distance_MeasPnt_Marker_Right[m]>"
  Reshape_306/1 -> SignalFilter/306
  Measurement_Points/3 -> Reshape_307/1  "<Velocity_MeasPnt_Marker_Left[m|s]>"
  Reshape_307/1 -> SignalFilter/307
  Measurement_Points/4 -> Reshape_308/1  "<Velocity_MeasPnt_Marker_Right[m|s]>"
  Reshape_308/1 -> SignalFilter/308
  Lane_Network/1 -> SignalFilter/309  "<LaneNetwork_State[]>"
  Lane_Network/2 -> DataTypeConversion_310/1  "<Data_Valid[]>"
  DataTypeConversion_310/1 -> SignalFilter/310
  Lane_Network/3 -> Reshape_311/1  "<LaneNetwork_Data[]>"
  Reshape_311/1 -> DataTypeConversion_311/1
  DataTypeConversion_311/1 -> SignalFilter/311
  Traffic_Signals_toEnvironment/1 -> Reshape_312/1  "<s_Fellows_Ref_Scheduler[m]>"
  Reshape_312/1 -> SignalFilter/312
  Traffic_Signals_toEnvironment/2 -> Reshape_313/1  "<d_Fellows_Ref_Scheduler[m]>"
  Reshape_313/1 -> SignalFilter/313
  Traffic_Signals_toEnvironment/3 -> Reshape_314/1  "<v_Fellows_Ref_Scheduler[km|h]>"
  Reshape_314/1 -> SignalFilter/314
  Traffic_Signals_toEnvironment/4 -> Reshape_315/1  "<LaneIdx_Fellows_Ref_Scheduler[]>"
  Reshape_315/1 -> SignalFilter/315
  Traffic_Signals_toEnvironment/5 -> Reshape_316/1  "<RelativeLane_Mode_Fellows[0CenterLane|1PreferredLane]>"
  Reshape_316/1 -> SignalFilter/316
  Traffic_Signals_toEnvironment/6 -> Reshape_317/1  "<ForceToRoad_Fellows_Ref_Scheduler[0|1]>"
  Reshape_317/1 -> SignalFilter/317
  Traffic_Signals_toEnvironment/7 -> Reshape_318/1  "<v_Lat_Fellows_Ref_Scheduler[m|s]>"
  Reshape_318/1 -> SignalFilter/318
  Traffic_Signals_toEnvironment/8 -> Reshape_319/1  "<Direction_Fellows_Ref_Scheduler[-1|1]>"
  Reshape_319/1 -> SignalFilter/319
  Traffic_Signals_toEnvironment/9 -> Reshape_320/1  "<Route_Id_Fellows_Ref_Scheduler[]>"
  Reshape_320/1 -> SignalFilter/320
  Traffic_Signals_toEnvironment/10 -> Reshape_321/1  "<Dist_Def_Trf[]>"
  Reshape_321/1 -> SignalFilter/321
  Traffic_Signals_toEnvironment/11 -> Reshape_322/1  "<Flag_FellowUsed[0|1]>"
  Reshape_322/1 -> SignalFilter/322
  Traffic_Signals_toEnvironment/12 -> SignalFilter/323  "<a_x_Vehicle_Ref[m|s2]>"
  Traffic_Signals_toEnvironment/13 -> SignalFilter/324  "<Dist_Refline_Response[m]>"
  Info1/1 -> SignalFilter/325  "<TrafficState[]>"
  Info1/2 -> SignalFilter/326  "<ErrorFlag[]>"
  Info1/3 -> Reshape_327/1  "<CurrentSequence_Fellows[]>"
  Reshape_327/1 -> SignalFilter/327
  Info1/4 -> Reshape_328/1  "<CurrentSegment_Fellows[]>"
  Reshape_328/1 -> SignalFilter/328
  Info1/5 -> Reshape_329/1  "<t_local_Fellows[s]>"
  Reshape_329/1 -> SignalFilter/329
  Info1/6 -> Reshape_330/1  "<CurrentSequence_UserSignals[]>"
  Reshape_330/1 -> SignalFilter/330
  Info1/7 -> Reshape_331/1  "<CurrentSegment_UserSignals[]>"
  Reshape_331/1 -> SignalFilter/331
  Info1/8 -> Reshape_332/1  "<t_local_UserSignals[s]>"
  Reshape_332/1 -> SignalFilter/332
  Info1/9 -> SignalFilter/333  "<CurrentSegment[]>"
  Info1/10 -> SignalFilter/334  "<t_local[s]>"
  Traffic_Signals_toEnvironment/15 -> Reshape_335/1  "<a_Fellows_Ref_Scheduler[m|s2]>"
  Reshape_335/1 -> SignalFilter/335
  Traffic_Signals_toEnvironment/16 -> Reshape_336/1  "<UserSignals_Fellows[]>"
  Reshape_336/1 -> SignalFilter/336
  Traffic_Signals_toEnvironment/17 -> Reshape_337/1  "<d_Total_Fellows[m]>"
  Reshape_337/1 -> SignalFilter/337
  Traffic_Signals_toEnvironment/18 -> Reshape_338/1  "<LaneIdx_Total_Fellows[]>"
  Reshape_338/1 -> SignalFilter/338
  Traffic_Signals_toEnvironment/19 -> Reshape_339/1  "<v_Fellows[km|h]>"
  Reshape_339/1 -> SignalFilter/339
  Pos_Fellows_MainPnt_CoorSys_E[x;y;z][m]/1 -> Reshape_340/1  "<Pos_x_Fellows[m]>"
  Reshape_340/1 -> SignalFilter/340
  Pos_Fellows_MainPnt_CoorSys_E[x;y;z][m]/2 -> Reshape_341/1  "<Pos_y_Fellows[m]>"
  Reshape_341/1 -> SignalFilter/341
  Pos_Fellows_MainPnt_CoorSys_E[x;y;z][m]/3 -> Reshape_342/1  "<Pos_z_Fellows[m]>"
  Reshape_342/1 -> SignalFilter/342
  Angle_Fellows[x;y;z][deg]/1 -> Reshape_343/1  "<Angle_Roll_Fellows[deg]>"
  Reshape_343/1 -> SignalFilter/343
  Angle_Fellows[x;y;z][deg]/2 -> Reshape_344/1  "<Angle_Pitch_Fellows[deg]>"
  Reshape_344/1 -> SignalFilter/344
  Angle_Fellows[x;y;z][deg]/3 -> Reshape_345/1  "<Angle_Yaw_Fellows[deg]>"
  Reshape_345/1 -> SignalFilter/345
  Angle_Fellows[x;y;z][deg]/4 -> Reshape_346/1  "<Angle_Wheel_Fellows[deg]>"
  Reshape_346/1 -> SignalFilter/346
  Traffic_Signals_toEnvironment/22 -> Reshape_347/1  "<Angle_Wheel_Fellows[deg]>"
  Reshape_347/1 -> SignalFilter/347
  Traffic_Signals_toEnvironment/23 -> Reshape_348/1  "<v_Fellows[x;y;z][km|h]>"
  Reshape_348/1 -> SignalFilter/348
  Traffic_Signals_toEnvironment/24 -> Reshape_349/1  "<w_Fellows[x;y;z][deg|s]>"
  Reshape_349/1 -> SignalFilter/349
  UserSignals_Customized2/1 -> SignalFilter/350  "<ManeuverSegmentEndTrigger[0|1]>"
  DriverMonitoring/1 -> SignalFilter/351  "<DriverGazeLocation[]>"
  DriverMonitoring/2 -> SignalFilter/352  "<DriverAnimation[]>"
  DriverMonitoring/3 -> SignalFilter/353  "<DriverLizardOwlRatio[]>"
  UserSignals_Customized2/3 -> Reshape_354/1  "<UserSignals>"
  Reshape_354/1 -> SignalFilter/354
  UserSignals_Customized2/4 -> SignalFilter/355  "<Fellow1_TurnLights>"
  UserSignals_Customized2/5 -> SignalFilter/356  "<Fellow2_TurnLights>"
  UserSignals_Customized2/6 -> SignalFilter/357  "<Fellow3_TurnLights>"
  UserSignals_Customized2/7 -> SignalFilter/358  "<Fellow4_TurnLights>"
  UserSignals_Customized2/8 -> SignalFilter/359  "<Fellow5_TurnLights>"
  UserSignals_Customized2/9 -> SignalFilter/360  "<Fellow6_TurnLights>"
  UserSignals_Customized2/10 -> SignalFilter/361  "<Fellow7_TurnLights>"
  UserSignals_Customized2/11 -> SignalFilter/362  "<Fellow8_TurnLights>"
  UserSignals_Customized2/12 -> SignalFilter/363  "<Fellow9_TurnLights>"
  UserSignals_Customized2/13 -> SignalFilter/364  "<Fellow10_TurnLights>"
  UserSignals_Customized2/14 -> SignalFilter/365  "<Fellow11_TurnLights>"
  UserSignals_Customized2/15 -> SignalFilter/366  "<Fellow12_TurnLights>"
  UserSignals_Customized2/16 -> SignalFilter/367  "<Fellow13_TurnLights>"
  UserSignals_Customized2/17 -> SignalFilter/368  "<Fellow14_TurnLights>"
  UserSignals_Customized2/18 -> SignalFilter/369  "<Fellow15_TurnLights>"
  UserSignals_Customized2/19 -> SignalFilter/370  "<Fellow16_TurnLights>"
  UserSignals_Customized2/20 -> SignalFilter/371  "<Fellow17_TurnLights>"
  UserSignals_Customized2/21 -> SignalFilter/372  "<Fellow18_TurnLights>"
  UserSignals_Customized2/22 -> SignalFilter/373  "<Fellow19_TurnLights>"
  UserSignals_Customized2/23 -> SignalFilter/374  "<Fellow20_TurnLights>"
  UserSignals_Customized2/24 -> SignalFilter/375  "<Fellow21_TurnLights>"
  UserSignals_Customized2/25 -> SignalFilter/376  "<Fellow22_TurnLights>"
  UserSignals_Customized2/26 -> SignalFilter/377  "<Fellow23_TurnLights>"
  UserSignals_Customized2/27 -> SignalFilter/378  "<Fellow24_TurnLights>"
  UserSignals_Customized2/28 -> SignalFilter/379  "<Fellow25_TurnLights>"
  UserSignals_Customized2/29 -> SignalFilter/380  "<Fellow26_TurnLights>"
  UserSignals_Customized2/30 -> SignalFilter/381  "<Fellow27_TurnLights>"
  UserSignals_Customized2/31 -> SignalFilter/382  "<Fellow28_TurnLights>"
  UserSignals_Customized2/32 -> SignalFilter/383  "<Fellow29_TurnLights>"
  UserSignals_Customized2/33 -> SignalFilter/384  "<Fellow30_TurnLights>"
  UserSignals_Customized2/34 -> SignalFilter/385  "<Fellow1_DoorFL>"
  UserSignals_Customized2/35 -> SignalFilter/386  "<Fellow2_DoorFL>"
  UserSignals_Customized2/36 -> SignalFilter/387  "<Fellow3_DoorFL>"
  UserSignals_Customized2/37 -> SignalFilter/388  "<Fellow4_DoorFL>"
  UserSignals_Customized2/38 -> SignalFilter/389  "<Fellow5_DoorFL>"
  UserSignals_Customized2/39 -> SignalFilter/390  "<Fellow6_DoorFL>"
  UserSignals_Customized2/40 -> SignalFilter/391  "<Fellow7_DoorFL>"
  UserSignals_Customized2/41 -> SignalFilter/392  "<Fellow8_DoorFL>"
  UserSignals_Customized2/42 -> SignalFilter/393  "<Fellow9_DoorFL>"
  UserSignals_Customized2/43 -> SignalFilter/394  "<Fellow10_DoorFL>"
  UserSignals_Customized2/44 -> SignalFilter/395  "<Fellow11_DoorFL>"
  UserSignals_Customized2/45 -> SignalFilter/396  "<Fellow12_DoorFL>"
  UserSignals_Customized2/46 -> SignalFilter/397  "<Fellow13_DoorFL>"
  UserSignals_Customized2/47 -> SignalFilter/398  "<Fellow14_DoorFL>"
  UserSignals_Customized2/48 -> SignalFilter/399  "<Fellow15_DoorFL>"
  UserSignals_Customized2/49 -> SignalFilter/400  "<Fellow16_DoorFL>"
  UserSignals_Customized2/50 -> SignalFilter/401  "<Fellow17_DoorFL>"
  UserSignals_Customized2/51 -> SignalFilter/402  "<Fellow18_DoorFL>"
  UserSignals_Customized2/52 -> SignalFilter/403  "<Fellow19_DoorFL>"
  UserSignals_Customized2/53 -> SignalFilter/404  "<Fellow20_DoorFL>"
  UserSignals_Customized2/54 -> SignalFilter/405  "<Fellow21_DoorFL>"
  UserSignals_Customized2/55 -> SignalFilter/406  "<Fellow22_DoorFL>"
  UserSignals_Customized2/56 -> SignalFilter/407  "<Fellow23_DoorFL>"
  UserSignals_Customized2/57 -> SignalFilter/408  "<Fellow24_DoorFL>"
  UserSignals_Customized2/58 -> SignalFilter/409  "<Fellow25_DoorFL>"
  UserSignals_Customized2/59 -> SignalFilter/410  "<Fellow26_DoorFL>"
  UserSignals_Customized2/60 -> SignalFilter/411  "<Fellow27_DoorFL>"
  UserSignals_Customized2/61 -> SignalFilter/412  "<Fellow28_DoorFL>"
  UserSignals_Customized2/62 -> SignalFilter/413  "<Fellow29_DoorFL>"
  UserSignals_Customized2/63 -> SignalFilter/414  "<Fellow30_DoorFL>"
  UserSignals_Customized2/64 -> SignalFilter/415  "<Fellow1_DoorFR>"
  UserSignals_Customized2/65 -> SignalFilter/416  "<Fellow2_DoorFR>"
  UserSignals_Customized2/66 -> SignalFilter/417  "<Fellow3_DoorFR>"
  UserSignals_Customized2/67 -> SignalFilter/418  "<Fellow4_DoorFR>"
  UserSignals_Customized2/68 -> SignalFilter/419  "<Fellow5_DoorFR>"
  UserSignals_Customized2/69 -> SignalFilter/420  "<Fellow6_DoorFR>"
  UserSignals_Customized2/70 -> SignalFilter/421  "<Fellow7_DoorFR>"
  UserSignals_Customized2/71 -> SignalFilter/422  "<Fellow8_DoorFR>"
  UserSignals_Customized2/72 -> SignalFilter/423  "<Fellow9_DoorFR>"
  UserSignals_Customized2/73 -> SignalFilter/424  "<Fellow10_DoorFR>"
  UserSignals_Customized2/74 -> SignalFilter/425  "<Fellow11_DoorFR>"
  UserSignals_Customized2/75 -> SignalFilter/426  "<Fellow12_DoorFR>"
  UserSignals_Customized2/76 -> SignalFilter/427  "<Fellow13_DoorFR>"
  UserSignals_Customized2/77 -> SignalFilter/428  "<Fellow14_DoorFR>"
  UserSignals_Customized2/78 -> SignalFilter/429  "<Fellow15_DoorFR>"
  UserSignals_Customized2/79 -> SignalFilter/430  "<Fellow16_DoorFR>"
  UserSignals_Customized2/80 -> SignalFilter/431  "<Fellow17_DoorFR>"
  UserSignals_Customized2/81 -> SignalFilter/432  "<Fellow18_DoorFR>"
  UserSignals_Customized2/82 -> SignalFilter/433  "<Fellow19_DoorFR>"
  UserSignals_Customized2/83 -> SignalFilter/434  "<Fellow20_DoorFR>"
  UserSignals_Customized2/84 -> SignalFilter/435  "<Fellow21_DoorFR>"
  UserSignals_Customized2/85 -> SignalFilter/436  "<Fellow22_DoorFR>"
  UserSignals_Customized2/86 -> SignalFilter/437  "<Fellow23_DoorFR>"
  UserSignals_Customized2/87 -> SignalFilter/438  "<Fellow24_DoorFR>"
  UserSignals_Customized2/88 -> SignalFilter/439  "<Fellow25_DoorFR>"
  UserSignals_Customized2/89 -> SignalFilter/440  "<Fellow26_DoorFR>"
  UserSignals_Customized2/90 -> SignalFilter/441  "<Fellow27_DoorFR>"
  UserSignals_Customized2/91 -> SignalFilter/442  "<Fellow28_DoorFR>"
  UserSignals_Customized2/92 -> SignalFilter/443  "<Fellow29_DoorFR>"
  UserSignals_Customized2/93 -> SignalFilter/444  "<Fellow30_DoorFR>"
  UserSignals_Customized2/94 -> SignalFilter/445  "<Fellow1_DoorRL>"
  UserSignals_Customized2/95 -> SignalFilter/446  "<Fellow2_DoorRL>"
  UserSignals_Customized2/96 -> SignalFilter/447  "<Fellow3_DoorRL>"
  UserSignals_Customized2/97 -> SignalFilter/448  "<Fellow4_DoorRL>"
  UserSignals_Customized2/98 -> SignalFilter/449  "<Fellow5_DoorRL>"
  UserSignals_Customized2/99 -> SignalFilter/450  "<Fellow6_DoorRL>"
  UserSignals_Customized2/100 -> SignalFilter/451  "<Fellow7_DoorRL>"
  UserSignals_Customized2/101 -> SignalFilter/452  "<Fellow8_DoorRL>"
  UserSignals_Customized2/102 -> SignalFilter/453  "<Fellow9_DoorRL>"
  UserSignals_Customized2/103 -> SignalFilter/454  "<Fellow10_DoorRL>"
  UserSignals_Customized2/104 -> SignalFilter/455  "<Fellow11_DoorRL>"
  UserSignals_Customized2/105 -> SignalFilter/456  "<Fellow12_DoorRL>"
  UserSignals_Customized2/106 -> SignalFilter/457  "<Fellow13_DoorRL>"
  UserSignals_Customized2/107 -> SignalFilter/458  "<Fellow14_DoorRL>"
  UserSignals_Customized2/108 -> SignalFilter/459  "<Fellow15_DoorRL>"
  UserSignals_Customized2/109 -> SignalFilter/460  "<Fellow16_DoorRL>"
  UserSignals_Customized2/110 -> SignalFilter/461  "<Fellow17_DoorRL>"
  UserSignals_Customized2/111 -> SignalFilter/462  "<Fellow18_DoorRL>"
  UserSignals_Customized2/112 -> SignalFilter/463  "<Fellow19_DoorRL>"
  UserSignals_Customized2/113 -> SignalFilter/464  "<Fellow20_DoorRL>"
  UserSignals_Customized2/114 -> SignalFilter/465  "<Fellow21_DoorRL>"
  UserSignals_Customized2/115 -> SignalFilter/466  "<Fellow22_DoorRL>"
  UserSignals_Customized2/116 -> SignalFilter/467  "<Fellow23_DoorRL>"
  UserSignals_Customized2/117 -> SignalFilter/468  "<Fellow24_DoorRL>"
  UserSignals_Customized2/118 -> SignalFilter/469  "<Fellow25_DoorRL>"
  UserSignals_Customized2/119 -> SignalFilter/470  "<Fellow26_DoorRL>"
  UserSignals_Customized2/120 -> SignalFilter/471  "<Fellow27_DoorRL>"
  UserSignals_Customized2/121 -> SignalFilter/472  "<Fellow28_DoorRL>"
  UserSignals_Customized2/122 -> SignalFilter/473  "<Fellow29_DoorRL>"
  UserSignals_Customized2/123 -> SignalFilter/474  "<Fellow30_DoorRL>"
  UserSignals_Customized2/124 -> SignalFilter/475  "<Fellow1_DoorRR>"
  UserSignals_Customized2/125 -> SignalFilter/476  "<Fellow2_DoorRR>"
  UserSignals_Customized2/126 -> SignalFilter/477  "<Fellow3_DoorRR>"
  UserSignals_Customized2/127 -> SignalFilter/478  "<Fellow4_DoorRR>"
  UserSignals_Customized2/128 -> SignalFilter/479  "<Fellow5_DoorRR>"
  UserSignals_Customized2/129 -> SignalFilter/480  "<Fellow6_DoorRR>"
  UserSignals_Customized2/130 -> SignalFilter/481  "<Fellow7_DoorRR>"
  UserSignals_Customized2/131 -> SignalFilter/482  "<Fellow8_DoorRR>"
  UserSignals_Customized2/132 -> SignalFilter/483  "<Fellow9_DoorRR>"
  UserSignals_Customized2/133 -> SignalFilter/484  "<Fellow10_DoorRR>"
  UserSignals_Customized2/134 -> SignalFilter/485  "<Fellow11_DoorRR>"
  UserSignals_Customized2/135 -> SignalFilter/486  "<Fellow12_DoorRR>"
  UserSignals_Customized2/136 -> SignalFilter/487  "<Fellow13_DoorRR>"
  UserSignals_Customized2/137 -> SignalFilter/488  "<Fellow14_DoorRR>"
  UserSignals_Customized2/138 -> SignalFilter/489  "<Fellow15_DoorRR>"
  UserSignals_Customized2/139 -> SignalFilter/490  "<Fellow16_DoorRR>"
  UserSignals_Customized2/140 -> SignalFilter/491  "<Fellow17_DoorRR>"
  UserSignals_Customized2/141 -> SignalFilter/492  "<Fellow18_DoorRR>"
  UserSignals_Customized2/142 -> SignalFilter/493  "<Fellow19_DoorRR>"
  UserSignals_Customized2/143 -> SignalFilter/494  "<Fellow20_DoorRR>"
  UserSignals_Customized2/144 -> SignalFilter/495  "<Fellow21_DoorRR>"
  UserSignals_Customized2/145 -> SignalFilter/496  "<Fellow22_DoorRR>"
  UserSignals_Customized2/146 -> SignalFilter/497  "<Fellow23_DoorRR>"
  UserSignals_Customized2/147 -> SignalFilter/498  "<Fellow24_DoorRR>"
  UserSignals_Customized2/148 -> SignalFilter/499  "<Fellow25_DoorRR>"
  UserSignals_Customized2/149 -> SignalFilter/500  "<Fellow26_DoorRR>"
  UserSignals_Customized2/150 -> SignalFilter/501  "<Fellow27_DoorRR>"
  UserSignals_Customized2/151 -> SignalFilter/502  "<Fellow28_DoorRR>"
  UserSignals_Customized2/152 -> SignalFilter/503  "<Fellow29_DoorRR>"
  UserSignals_Customized2/153 -> SignalFilter/504  "<Fellow30_DoorRR>"
  UserSignals_Customized2/154 -> SignalFilter/505  "<Fellow1_Hood>"
  UserSignals_Customized2/155 -> SignalFilter/506  "<Fellow2_Hood>"
  UserSignals_Customized2/156 -> SignalFilter/507  "<Fellow3_Hood>"
  UserSignals_Customized2/157 -> SignalFilter/508  "<Fellow4_Hood>"
  UserSignals_Customized2/158 -> SignalFilter/509  "<Fellow5_Hood>"
  UserSignals_Customized2/159 -> SignalFilter/510  "<Fellow6_Hood>"
  UserSignals_Customized2/160 -> SignalFilter/511  "<Fellow7_Hood>"
  UserSignals_Customized2/161 -> SignalFilter/512  "<Fellow8_Hood>"
  UserSignals_Customized2/162 -> SignalFilter/513  "<Fellow9_Hood>"
  UserSignals_Customized2/163 -> SignalFilter/514  "<Fellow10_Hood>"
  UserSignals_Customized2/164 -> SignalFilter/515  "<Fellow11_Hood>"
  UserSignals_Customized2/165 -> SignalFilter/516  "<Fellow12_Hood>"
  UserSignals_Customized2/166 -> SignalFilter/517  "<Fellow13_Hood>"
  UserSignals_Customized2/167 -> SignalFilter/518  "<Fellow14_Hood>"
  UserSignals_Customized2/168 -> SignalFilter/519  "<Fellow15_Hood>"
  UserSignals_Customized2/169 -> SignalFilter/520  "<Fellow16_Hood>"
  UserSignals_Customized2/170 -> SignalFilter/521  "<Fellow17_Hood>"
  UserSignals_Customized2/171 -> SignalFilter/522  "<Fellow18_Hood>"
  UserSignals_Customized2/172 -> SignalFilter/523  "<Fellow19_Hood>"
  UserSignals_Customized2/173 -> SignalFilter/524  "<Fellow20_Hood>"
  UserSignals_Customized2/174 -> SignalFilter/525  "<Fellow21_Hood>"
  UserSignals_Customized2/175 -> SignalFilter/526  "<Fellow22_Hood>"
  UserSignals_Customized2/176 -> SignalFilter/527  "<Fellow23_Hood>"
  UserSignals_Customized2/177 -> SignalFilter/528  "<Fellow24_Hood>"
  UserSignals_Customized2/178 -> SignalFilter/529  "<Fellow25_Hood>"
  UserSignals_Customized2/179 -> SignalFilter/530  "<Fellow26_Hood>"
  UserSignals_Customized2/180 -> SignalFilter/531  "<Fellow27_Hood>"
  UserSignals_Customized2/181 -> SignalFilter/532  "<Fellow28_Hood>"
  UserSignals_Customized2/182 -> SignalFilter/533  "<Fellow29_Hood>"
  UserSignals_Customized2/183 -> SignalFilter/534  "<Fellow30_Hood>"
  UserSignals_Customized2/184 -> SignalFilter/535  "<Fellow1_Trunk>"
  UserSignals_Customized2/185 -> SignalFilter/536  "<Fellow2_Trunk>"
  UserSignals_Customized2/186 -> SignalFilter/537  "<Fellow3_Trunk>"
  UserSignals_Customized2/187 -> SignalFilter/538  "<Fellow4_Trunk>"
  UserSignals_Customized2/188 -> SignalFilter/539  "<Fellow5_Trunk>"
  UserSignals_Customized2/189 -> SignalFilter/540  "<Fellow6_Trunk>"
  UserSignals_Customized2/190 -> SignalFilter/541  "<Fellow7_Trunk>"
  UserSignals_Customized2/191 -> SignalFilter/542  "<Fellow8_Trunk>"
  UserSignals_Customized2/192 -> SignalFilter/543  "<Fellow9_Trunk>"
  UserSignals_Customized2/193 -> SignalFilter/544  "<Fellow10_Trunk>"
  UserSignals_Customized2/194 -> SignalFilter/545  "<Fellow11_Trunk>"
  UserSignals_Customized2/195 -> SignalFilter/546  "<Fellow12_Trunk>"
  UserSignals_Customized2/196 -> SignalFilter/547  "<Fellow13_Trunk>"
  UserSignals_Customized2/197 -> SignalFilter/548  "<Fellow14_Trunk>"
  UserSignals_Customized2/198 -> SignalFilter/549  "<Fellow15_Trunk>"
  UserSignals_Customized2/199 -> SignalFilter/550  "<Fellow16_Trunk>"
  UserSignals_Customized2/200 -> SignalFilter/551  "<Fellow17_Trunk>"
  UserSignals_Customized2/201 -> SignalFilter/552  "<Fellow18_Trunk>"
  UserSignals_Customized2/202 -> SignalFilter/553  "<Fellow19_Trunk>"
  UserSignals_Customized2/203 -> SignalFilter/554  "<Fellow20_Trunk>"
  UserSignals_Customized2/204 -> SignalFilter/555  "<Fellow21_Trunk>"
  UserSignals_Customized2/205 -> SignalFilter/556  "<Fellow22_Trunk>"
  UserSignals_Customized2/206 -> SignalFilter/557  "<Fellow23_Trunk>"
  UserSignals_Customized2/207 -> SignalFilter/558  "<Fellow24_Trunk>"
  UserSignals_Customized2/208 -> SignalFilter/559  "<Fellow25_Trunk>"
  UserSignals_Customized2/209 -> SignalFilter/560  "<Fellow26_Trunk>"
  UserSignals_Customized2/210 -> SignalFilter/561  "<Fellow27_Trunk>"
  UserSignals_Customized2/211 -> SignalFilter/562  "<Fellow28_Trunk>"
  UserSignals_Customized2/212 -> SignalFilter/563  "<Fellow29_Trunk>"
  UserSignals_Customized2/213 -> SignalFilter/564  "<Fellow30_Trunk>"
  Control/1 -> SignalFilter/565  "<Quadrant_Def_Mode[1Internal|2External]>"
  Control/2 -> SignalFilter/566  "<Quadrant_Dim_x[m]>"
  Control/3 -> SignalFilter/567  "<Quadrant_Dim_y[m]>"
  Control/4 -> SignalFilter/568  "<Interface_Mode[0Off|1ObjOnly|2ObjAndLanes]>"
  Control/5 -> SignalFilter/569  "<Interface_Init[0Off|1On]>"
  Control/6 -> SignalFilter/570  "<Interface_Init_Ready[0Off|1On]>"
  FellowSignalLabels/1 -> Reshape_571/1  "<d_Total_Fellows[m]>"
  Reshape_571/1 -> SignalFilter/571
  FellowSignalLabels/2 -> Reshape_572/1  "<LaneIdx_Total_Fellows[]>"
  Reshape_572/1 -> SignalFilter/572
  FellowSignalLabels/3 -> Reshape_573/1  "<s_Fellows[m]>"
  Reshape_573/1 -> SignalFilter/573
  FellowSignalLabels/4 -> Reshape_574/1  "<v_Fellows[km|h]>"
  Reshape_574/1 -> SignalFilter/574
  Info2/1 -> SignalFilter/575  "<FellowParameters_Sfcn_State[]>"
  Info2/2 -> SignalFilter/576  "<FellowParameters_Data_Valid[0|1]>"
  FellowParameters/2 -> Reshape_577/1  "<Data_Valid_Fellows[0|1]>"
  Reshape_577/1 -> SignalFilter/577
  FellowParameters/3 -> Reshape_578/1  "<PosVec_MainPnt_Fellows[x;y;z][m]>"
  Reshape_578/1 -> SignalFilter/578
  FellowParameters/4 -> Reshape_579/1  "<Length_Fellows[m]>"
  Reshape_579/1 -> SignalFilter/579
  FellowParameters/5 -> Reshape_580/1  "<Width_Fellows[m]>"
  Reshape_580/1 -> SignalFilter/580
  FellowParameters/6 -> Reshape_581/1  "<Height_Fellows[m]>"
  Reshape_581/1 -> SignalFilter/581
  FellowParameters/7 -> Reshape_582/1  "<Wheel_Radius_Fellows[m]>"
  Reshape_582/1 -> SignalFilter/582
  FellowParameters/8 -> Reshape_583/1  "<TrackWidth_Front_Fellows[m]>"
  Reshape_583/1 -> SignalFilter/583
  FellowParameters/9 -> Reshape_584/1  "<TrackWidth_Rear_Fellows[m]>"
  Reshape_584/1 -> SignalFilter/584
  FellowParameters/10 -> Reshape_585/1  "<WheelBase_Fellows[m]>"
  Reshape_585/1 -> SignalFilter/585
  FellowParameters/11 -> Reshape_586/1  "<TrafficObject_Type_Fellows[]>"
  Reshape_586/1 -> SignalFilter/586
  FellowParameters/12 -> Reshape_587/1  "<Movement_Characteristics[]>"
  Reshape_587/1 -> DataTypeConversion_587/1
  DataTypeConversion_587/1 -> SignalFilter/587
  FellowParameters/13 -> Reshape_588/1  "<Hitch_Dist[m]>"
  Reshape_588/1 -> SignalFilter/588
  TrafficObjects/1 -> SignalFilter/589  "<Flag_TrafficObject_Init_Ready[0|1]>"
  TrafficObjects/2 -> SignalFilter/590  "<TrafficObjectsState[]>"
  TrafficObjects/3 -> DataTypeConversion_591/1  "<Data_Valid[]>"
  DataTypeConversion_591/1 -> SignalFilter/591
  TrafficObjects/4 -> Reshape_592/1  "<TrafficObject_Type_Data[]>"
  Reshape_592/1 -> DataTypeConversion_592/1
  DataTypeConversion_592/1 -> SignalFilter/592
  DiscreteObjects/1 -> SignalFilter/593  "<Flag_DiscreteObject_Init_Ready[0|1]>"
  DiscreteObjects/2 -> SignalFilter/594  "<DiscreteObjectsState[]>"
  DiscreteObjects/3 -> DataTypeConversion_595/1  "<Data_Valid[]>"
  DataTypeConversion_595/1 -> SignalFilter/595
  DiscreteObjects/4 -> Reshape_596/1  "<DiscreteObject_Data[]>"
  Reshape_596/1 -> DataTypeConversion_596/1
  DataTypeConversion_596/1 -> SignalFilter/596
  Control1/1 -> SignalFilter/597  "<Quadrant_Def_Mode[1Internal|2External]>"
  Control1/2 -> SignalFilter/598  "<Quadrant_Dim_x[m]>"
  Control1/3 -> SignalFilter/599  "<Quadrant_Dim_y[m]>"
  Control1/4 -> SignalFilter/600  "<Interface_Mode[0Off|1ObjOnly|2ObjAndLanes]>"
  Control1/5 -> SignalFilter/601  "<Interface_Init[0Off|1On]>"
  Control1/6 -> SignalFilter/602  "<Interface_Init_Ready[0Off|1On]>"
  Info3/1 -> SignalFilter/603  "<Interface_State[]>"
  Data/1 -> Reshape_604/1  "<GroundTruth_Interface_Data[]>"
  Reshape_604/1 -> DataTypeConversion_604/1
  DataTypeConversion_604/1 -> SignalFilter/604
  Data/2 -> Reshape_605/1  "<HostVehicle_Data>"
  Reshape_605/1 -> DataTypeConversion_605/1
  DataTypeConversion_605/1 -> SignalFilter/605
  Data_Access/1 -> SignalFilter/606  "<Num_MovObj[]>"
  Data_Access/2 -> SignalFilter/607  "<Num_MovObj_in_GT_Area[]>"
  Data_Access/3 -> SignalFilter/608  "<Num_StatObj[]>"
  Data_Access/4 -> SignalFilter/609  "<Num_StatObj_in_GT_Area[]>"
  Data_Access/5 -> SignalFilter/610  "<Num_Laneboundaries[]>"
  Data_Access/6 -> SignalFilter/611  "<Num_Lanes[]>"
  Data_Access/7 -> SignalFilter/612  "<Num_TrfLights[]>"
  Data_Access/8 -> SignalFilter/613  "<Num_TrfLights_in_GT_Area[]>"
  Data_Access/9 -> SignalFilter/614  "<Num_TrfSigns[]>"
  Data_Access/10 -> SignalFilter/615  "<Num_TrfSigns_in_GT_Area[]>"
  OpenSimulationInterface/1 -> Reshape_616/1  "<MovObj_Type[]>"
  Reshape_616/1 -> SignalFilter/616
  OpenSimulationInterface/2 -> Reshape_617/1  "<MovObj_Vehicle_Type[]>"
  Reshape_617/1 -> SignalFilter/617
  OpenSimulationInterface/3 -> Reshape_618/1  "<MovObj_ID[]>"
  Reshape_618/1 -> SignalFilter/618
  OpenSimulationInterface/4 -> Reshape_619/1  "<MovObj_Position_x[m]>"
  Reshape_619/1 -> SignalFilter/619
  OpenSimulationInterface/5 -> Reshape_620/1  "<MovObj_Position_y[m]>"
  Reshape_620/1 -> SignalFilter/620
  OpenSimulationInterface/6 -> Reshape_621/1  "<MovObj_Position_z[m]>"
  Reshape_621/1 -> SignalFilter/621
  OpenSimulationInterface/7 -> Reshape_622/1  "<MovObj_Orientation_x[deg]>"
  Reshape_622/1 -> SignalFilter/622
  OpenSimulationInterface/8 -> Reshape_623/1  "<MovObj_Orientation_y[deg]>"
  Reshape_623/1 -> SignalFilter/623
  OpenSimulationInterface/9 -> Reshape_624/1  "<MovObj_Orientation_z[deg]>"
  Reshape_624/1 -> SignalFilter/624
  OpenSimulationInterface/10 -> Reshape_625/1  "<MovObj_Length[m]>"
  Reshape_625/1 -> SignalFilter/625
  OpenSimulationInterface/11 -> Reshape_626/1  "<MovObj_Width[m]>"
  Reshape_626/1 -> SignalFilter/626
  OpenSimulationInterface/12 -> Reshape_627/1  "<MovObj_Height[m]>"
  Reshape_627/1 -> SignalFilter/627
  Info4/1 -> SignalFilter/628  "<Sfunc_State[]>"
  Info4/2 -> SignalFilter/629  "<Data_Valid[0|1]>"
  Info4/3 -> SignalFilter/630  "<Flag_Sensor_Init_Ready[0|1]>"
  SensorOutput/1 -> SignalFilter/631  "<Collision_Flag[0NoCollision|1Collision]>"
  SensorOutput/2 -> SignalFilter/632  "<Collision_Flag_Held[0NoCollision|1Collision]>"
  SensorOutput/3 -> Reshape_633/1  "<Object_ID[]>"
  Reshape_633/1 -> SignalFilter/633
  SensorOutput/4 -> Reshape_634/1  "<Time_Collision[s]>"
  Reshape_634/1 -> SignalFilter/634
  SensorOutput/5 -> Reshape_635/1  "<Pos_Collision_Point[x;y][m]>"
  Reshape_635/1 -> SignalFilter/635
  SensorOutput/6 -> Reshape_636/1  "<v_Collision_CoG_Vehicle[x;y][m|s]>"
  Reshape_636/1 -> SignalFilter/636
  SensorOutput/7 -> Reshape_637/1  "<v_Collision_CoG_Vehicle_Total[m|s]>"
  Reshape_637/1 -> SignalFilter/637
  SensorOutput/8 -> Reshape_638/1  "<v_Rel_Collision_Point[x;y][m|s]>"
  Reshape_638/1 -> SignalFilter/638
  SensorOutput/9 -> Reshape_639/1  "<v_Rel_Collision_Point_Total[m|s]>"
  Reshape_639/1 -> SignalFilter/639
  Info5/1 -> SignalFilter/640  "<TrafficSignSensor_Dyn_Sfcn_State[]>"
  Info5/2 -> SignalFilter/641  "<TrafficSignSensor_Dyn_Data_Valid[0|1]>"
  SensorOutput[]/1 -> Reshape_642/1  "<Traffic_Sign_Valid[0|1]>"
  Reshape_642/1 -> SignalFilter/642
  SensorOutput[]/2 -> Reshape_643/1  "<TrafficObject_ID[]>"
  Reshape_643/1 -> SignalFilter/643
  SensorOutput[]/3 -> Reshape_644/1  "<TrafficObject_Type[]>"
  Reshape_644/1 -> SignalFilter/644
  SensorOutput[]/4 -> Reshape_645/1  "<Pos_CoorSys_E[x;y;z][m]>"
  Reshape_645/1 -> SignalFilter/645
  SensorOutput[]/5 -> Reshape_646/1  "<Angle_CoorSys_E[x;y;z][deg]>"
  Reshape_646/1 -> SignalFilter/646
  SensorOutput[]/6 -> Reshape_647/1  "<Pos_CoorSys_S[x;y;z][m]>"
  Reshape_647/1 -> SignalFilter/647
  SensorOutput[]/7 -> Reshape_648/1  "<Angle_Hor_Rel[deg]>"
  Reshape_648/1 -> SignalFilter/648
  SensorOutput[]/8 -> Reshape_649/1  "<Angle_Ver_Rel[deg]>"
  Reshape_649/1 -> SignalFilter/649
  SensorOutput[]/9 -> Reshape_650/1  "<Angle_Sign_Orientation_Rel[deg]>"
  Reshape_650/1 -> SignalFilter/650
  SensorOutput[]/10 -> Reshape_651/1  "<Distance[m]>"
  Reshape_651/1 -> SignalFilter/651
  SensorOutput[]/11 -> Reshape_652/1  "<Traffic_Sign_Type[]>"
  Reshape_652/1 -> SignalFilter/652
  SensorOutput[]/12 -> Reshape_653/1  "<Traffic_Sign_Subtype[]>"
  Reshape_653/1 -> SignalFilter/653
  SensorOutput[]/13 -> Reshape_654/1  "<Traffic_Sign_Value[]>"
  Reshape_654/1 -> SignalFilter/654
  SensorOutput[]/14 -> Reshape_655/1  "<Traffic_Sign_Country[]>"
  Reshape_655/1 -> SignalFilter/655
  SensorOutput[]/15 -> Reshape_656/1  "<Traffic_Sign_Visibility[0_100]>"
  Reshape_656/1 -> SignalFilter/656
  SensorOutput[]/16 -> Reshape_657/1  "<Traffic_Sign_Lanes[]>"
  Reshape_657/1 -> SignalFilter/657
  SensorOutput[]/17 -> Reshape_658/1  "<Object_Stream_ID[]>"
  Reshape_658/1 -> SignalFilter/658
  SensorOutput[]/18 -> Reshape_659/1  "<Object_State[]>"
  Reshape_659/1 -> SignalFilter/659
  SensorOutput[]/19 -> Reshape_660/1  "<Parent_Object_ID[]>"
  Reshape_660/1 -> SignalFilter/660
  SensorOutput[]/20 -> Reshape_661/1  "<Network_Item_Type[0Junction|1Road]>"
  Reshape_661/1 -> SignalFilter/661
  SensorOutput[]/21 -> Reshape_662/1  "<Network_Item_ID[]>"
  Reshape_662/1 -> SignalFilter/662
  Parameters2/1 -> SignalFilter/663  "<Sensor_Enable[0Off|1On]>"
  Parameters2/2 -> Reshape_664/1  "<Pos_Sensor_Apex_CoorSys_V[x;y;z][m]>"
  Reshape_664/1 -> SignalFilter/664
  Parameters2/3 -> Reshape_665/1  "<Angle_Orientation_Sensor_CoorSys_V[x;y;z][deg]>"
  Reshape_665/1 -> SignalFilter/665
  Parameters2/4 -> SignalFilter/666  "<Length_ScopeZone[m]>"
  Parameters2/5 -> SignalFilter/667  "<Angle_ScopeZone_Horizontal[deg]>"
  Parameters2/6 -> SignalFilter/668  "<Angle_ScopeZone_Vertical[deg]>"
  Parameters2/7 -> SignalFilter/669  "<Angle_Sign_Orientation_Max[deg]>"
  Parameter/1 -> SignalFilter/670  "<Sensor_Enable[0Off|1On]>"
  Parameter/2 -> SignalFilter/671  "<SensorIdx[]>"
  Parameter/3 -> SignalFilter/672  "<t_Offs_Sensor[s]>"
  Parameter/4 -> SignalFilter/673  "<t_Cycle_Sensor[s]>"
  Parameter/5 -> SignalFilter/674  "<t_Delay_SensorOutput[s]>"
  Parameter/6 -> SignalFilter/675  "<Geometry[]>"
  Parameter/7 -> Reshape_676/1  "<Pos_Sensor_Apex_CoorSys_V[x;y;z][m]>"
  Reshape_676/1 -> SignalFilter/676
  Parameter/8 -> Reshape_677/1  "<Angle_Orientation_Sensor_CoorSys_V[x;y;z][deg]>"
  Reshape_677/1 -> SignalFilter/677
  Parameter/9 -> SignalFilter/678  "<Length_ScopeZone[m]>"
  Parameter/10 -> SignalFilter/679  "<Angle_ScopeZone_Horizontal[deg]>"
  Parameter/11 -> SignalFilter/680  "<Angle_ScopeZone_Vertical[deg]>"
  Parameter/12 -> SignalFilter/681  "<Length_ScopeZone_Head[m]>"
  Parameter/13 -> SignalFilter/682  "<Length_BlindZone[m]>"
  Parameter/14 -> SignalFilter/683  "<Occlusion_Mode[1No_Occlusion|2Basic_3D|3Occlusion_Ratio_3D]>"
  Parameter/15 -> SignalFilter/684  "<Threshold_Occlusion_Ratio[0_1]>"
  Parameter/16 -> SignalFilter/685  "<Object_Points_Calculation_Enable[0Off|1On]>"
  Parameter/17 -> SignalFilter/686  "<Object_Points_Occlusion_Enable[0Off|1On]>"
  SensorIndex/1 -> SignalFilter/687  "<Idx_Sensor[]>"
  Info6/1 -> Reshape_688/1  "<Flag_Object_In_Scope[0Out|1In]>"
  Reshape_688/1 -> SignalFilter/688
  Info6/2 -> Reshape_689/1  "<Flag_Sensor_Apex_In_Object[0Out|1In]>"
  Reshape_689/1 -> SignalFilter/689
  Info6/3 -> SignalFilter/690  "<ObjectSensor3D_Sfcn_State[]>"
  Info6/4 -> SignalFilter/691  "<ObjectSensor3D_Data_Valid[0|1]>"
  Info6/5 -> SignalFilter/692  "<Flag_Sensor_Init_Ready[0|1]>"
  SensorOutput1/1 -> Reshape_693/1  "<v_Rel_Object[m|s]>"
  Reshape_693/1 -> SignalFilter/693
  SensorOutput1/2 -> Reshape_694/1  "<v_Object_CoorSys_S[x;y;z][m|s]>"
  Reshape_694/1 -> SignalFilter/694
  SensorOutput1/3 -> Reshape_695/1  "<a_Rel_Object[m|s2]>"
  Reshape_695/1 -> SignalFilter/695
  SensorOutput1/4 -> Reshape_696/1  "<a_Object_CoorSys_S[x;y;z][m|s2]>"
  Reshape_696/1 -> SignalFilter/696
  SensorOutput1/5 -> Reshape_697/1  "<Dist_Object[m]>"
  Reshape_697/1 -> SignalFilter/697
  SensorOutput1/6 -> Reshape_698/1  "<Angle_Hor_Object[deg]>"
  Reshape_698/1 -> SignalFilter/698
  SensorOutput1/7 -> Reshape_699/1  "<Angle_Ver_Object[deg]>"
  Reshape_699/1 -> SignalFilter/699
  SensorOutput1/8 -> Reshape_700/1  "<Pos_Sensor_Apex_E[x;y;z][m]>"
  Reshape_700/1 -> SignalFilter/700
  SensorOutput1/9 -> Reshape_701/1  "<Pos_Object_NearestPnt_S[x;y;z][m]>"
  Reshape_701/1 -> SignalFilter/701
  SensorOutput1/10 -> Reshape_702/1  "<Pos_Object_NearestPnt_E[x;y;z][m]>"
  Reshape_702/1 -> SignalFilter/702
  SensorOutput1/11 -> Reshape_703/1  "<Object_Info[-1None|1Fellow|2Static]>"
  Reshape_703/1 -> SignalFilter/703
  SensorOutput1/12 -> Reshape_704/1  "<Object_ID[]>"
  Reshape_704/1 -> SignalFilter/704
  SensorOutput1/13 -> Reshape_705/1  "<Object_Type[]>"
  Reshape_705/1 -> SignalFilter/705
  SensorOutput1/14 -> Reshape_706/1  "<Object_Age[s]>"
  Reshape_706/1 -> SignalFilter/706
  SensorOutput1/15 -> Reshape_707/1  "<Object_In_Scope_Entry_First[s]>"
  Reshape_707/1 -> SignalFilter/707
  SensorOutput1/16 -> Reshape_708/1  "<Object_In_Scope_Entry_Number[]>"
  Reshape_708/1 -> SignalFilter/708
  SensorOutput1/17 -> Reshape_709/1  "<Occlusion_Ratio_Object[-1|0_1]>"
  Reshape_709/1 -> SignalFilter/709
  SensorOutput1/18 -> Reshape_710/1  "<Flag_NearestPnt_Occluded[-1|0|1]>"
  Reshape_710/1 -> SignalFilter/710
  SensorOutput1/19 -> Reshape_711/1  "<Pos_NearestSurf_Pnt1_CoorSys_S[x;y;z][m]>"
  Reshape_711/1 -> SignalFilter/711
  SensorOutput1/20 -> Reshape_712/1  "<Pos_NearestSurf_Pnt2_CoorSys_S[x;y;z][m]>"
  Reshape_712/1 -> SignalFilter/712
  SensorOutput1/21 -> Reshape_713/1  "<Pos_NearestSurf_Pnt3_CoorSys_S[x;y;z][m]>"
  Reshape_713/1 -> SignalFilter/713
  SensorOutput1/22 -> Reshape_714/1  "<Pos_NearestSurf_Pnt4_CoorSys_S[x;y;z][m]>"
  Reshape_714/1 -> SignalFilter/714
  SensorOutput1/23 -> Reshape_715/1  "<NearestSurf_Pnts_Index[]>"
  Reshape_715/1 -> SignalFilter/715
  SensorOutput1/24 -> Reshape_716/1  "<NearestSurf_Index[]>"
  Reshape_716/1 -> SignalFilter/716
  SensorTimeStamp/1 -> SignalFilter/717  "<ObjectSample[s]>"
  SensorTimeStamp/2 -> SignalFilter/718  "<SensorCalculation[s]>"
  RadarEffects/1 -> Reshape_719/1  "<ID[]>"
  Reshape_719/1 -> SignalFilter/719
  RadarEffects/2 -> Reshape_720/1  "<Object_ID[]>"
  Reshape_720/1 -> SignalFilter/720
  RadarEffects/3 -> Reshape_721/1  "<Dist_CoorSys_S[m]>"
  Reshape_721/1 -> SignalFilter/721
  RadarEffects/4 -> Reshape_722/1  "<Angle_Hor_CoorSys_S[deg]>"
  Reshape_722/1 -> SignalFilter/722
  RadarEffects/5 -> Reshape_723/1  "<Pos_ObjectPoint_CoorSys_E[x;y;z][m]>"
  Reshape_723/1 -> SignalFilter/723
  CustomPoints/1 -> Reshape_724/1  "<ID[]>"
  Reshape_724/1 -> SignalFilter/724
  CustomPoints/2 -> Reshape_725/1  "<Object_ID[]>"
  Reshape_725/1 -> SignalFilter/725
  CustomPoints/3 -> Reshape_726/1  "<Dist_CoorSys_S[m]>"
  Reshape_726/1 -> SignalFilter/726
  CustomPoints/4 -> Reshape_727/1  "<Angle_Hor_CoorSys_S[deg]>"
  Reshape_727/1 -> SignalFilter/727
  CustomPoints/5 -> Reshape_728/1  "<Pos_CoorSys_E[x;y;z][m]>"
  Reshape_728/1 -> SignalFilter/728
  Object_Positions/1 -> Reshape_729/1  "<Pos_x_MainPnt_Objects_CoorSysE[m]>"
  Reshape_729/1 -> SignalFilter/729
  Object_Positions/2 -> Reshape_730/1  "<Pos_y_MainPnt_Objects_CoorSysE[m]>"
  Reshape_730/1 -> SignalFilter/730
  Object_Positions/3 -> Reshape_731/1  "<Pos_z_MainPnt_Objects_CoorSysE[m]>"
  Reshape_731/1 -> SignalFilter/731
  Object_Positions/4 -> Reshape_732/1  "<Angle_x_Objects_CoorSysE[deg]>"
  Reshape_732/1 -> SignalFilter/732
  Object_Positions/5 -> Reshape_733/1  "<Angle_y_Objects_CoorSysE[deg]>"
  Reshape_733/1 -> SignalFilter/733
  Object_Positions/6 -> Reshape_734/1  "<Angle_z_Objects_CoorSysE[deg]>"
  Reshape_734/1 -> SignalFilter/734
  Object_Positions/7 -> Reshape_735/1  "<Network_Item_Type[]>"
  Reshape_735/1 -> SignalFilter/735
  Object_Positions/8 -> Reshape_736/1  "<Network_Item_Id[]>"
  Reshape_736/1 -> SignalFilter/736
  Object_Positions/9 -> Reshape_737/1  "<Object_ID[]>"
  Reshape_737/1 -> SignalFilter/737
  Object_Properties_Box/1 -> Reshape_738/1  "<Flag_BoxProperties[0|1]>"
  Reshape_738/1 -> SignalFilter/738
  Object_Properties_Box/2 -> Reshape_739/1  "<PosVec_x_CenterPnt_Object[m]>"
  Reshape_739/1 -> SignalFilter/739
  Object_Properties_Box/3 -> Reshape_740/1  "<PosVec_y_CenterPnt_Object[m]>"
  Reshape_740/1 -> SignalFilter/740
  Object_Properties_Box/4 -> Reshape_741/1  "<PosVec_z_CenterPnt_Object[m]>"
  Reshape_741/1 -> SignalFilter/741
  Object_Properties_Box/5 -> Reshape_742/1  "<Length_Object[m]>"
  Reshape_742/1 -> SignalFilter/742
  Object_Properties_Box/6 -> Reshape_743/1  "<Width_Object[m]>"
  Reshape_743/1 -> SignalFilter/743
  Object_Properties_Box/7 -> Reshape_744/1  "<Height_Object[m]>"
  Reshape_744/1 -> SignalFilter/744
  Object_Properties_Box/8 -> Reshape_745/1  "<Object_Type[]>"
  Reshape_745/1 -> SignalFilter/745
  Object_Custom_Values/1 -> Reshape_746/1  "<Object_Valid[0|1]>"
  Reshape_746/1 -> SignalFilter/746
  Object_Custom_Values/2 -> Reshape_747/1  "<CustomValues[]>"
  Reshape_747/1 -> SignalFilter/747
  Parameter1/1 -> SignalFilter/748  "<Sensor_Enable[0Off|1On]>"
  Parameter1/2 -> SignalFilter/749  "<SensorIdx[]>"
  Parameter1/3 -> SignalFilter/750  "<t_Offs_Sensor[s]>"
  Parameter1/4 -> SignalFilter/751  "<t_Cycle_Sensor[s]>"
  Parameter1/5 -> SignalFilter/752  "<t_Delay_SensorOutput[s]>"
  Parameter1/6 -> SignalFilter/753  "<Geometry[]>"
  Parameter1/7 -> Reshape_754/1  "<Pos_Sensor_Apex_CoorSys_V[x;y;z][m]>"
  Reshape_754/1 -> SignalFilter/754
  Parameter1/8 -> Reshape_755/1  "<Angle_Orientation_Sensor_CoorSys_V[x;y;z][deg]>"
  Reshape_755/1 -> SignalFilter/755
  Parameter1/9 -> SignalFilter/756  "<Length_ScopeZone[m]>"
  Parameter1/10 -> SignalFilter/757  "<Angle_ScopeZone_Horizontal[deg]>"
  Parameter1/11 -> SignalFilter/758  "<Angle_ScopeZone_Vertical[deg]>"
  Parameter1/12 -> SignalFilter/759  "<Length_ScopeZone_Head[m]>"
  Parameter1/13 -> SignalFilter/760  "<Length_BlindZone[m]>"
  Parameter1/14 -> SignalFilter/761  "<Occlusion_Mode[1No_Occlusion|2Basic_3D|3Occlusion_Ratio_3D]>"
  Parameter1/15 -> SignalFilter/762  "<Threshold_Occlusion_Ratio[0_1]>"
  Parameter1/16 -> SignalFilter/763  "<Object_Points_Calculation_Enable[0Off|1On]>"
  Parameter1/17 -> SignalFilter/764  "<Object_Points_Occlusion_Enable[0Off|1On]>"
  SensorIndex1/1 -> SignalFilter/765  "<Idx_Sensor[]>"
  Info7/1 -> Reshape_766/1  "<Flag_Object_In_Scope[0Out|1In]>"
  Reshape_766/1 -> SignalFilter/766
  Info7/2 -> Reshape_767/1  "<Flag_Sensor_Apex_In_Object[0Out|1In]>"
  Reshape_767/1 -> SignalFilter/767
  Info7/3 -> SignalFilter/768  "<ObjectSensor3D_Sfcn_State[]>"
  Info7/4 -> SignalFilter/769  "<ObjectSensor3D_Data_Valid[0|1]>"
  Info7/5 -> SignalFilter/770  "<Flag_Sensor_Init_Ready[0|1]>"
  SensorOutput2/1 -> Reshape_771/1  "<v_Rel_Object[m|s]>"
  Reshape_771/1 -> SignalFilter/771
  SensorOutput2/2 -> Reshape_772/1  "<v_Object_CoorSys_S[x;y;z][m|s]>"
  Reshape_772/1 -> SignalFilter/772
  SensorOutput2/3 -> Reshape_773/1  "<a_Rel_Object[m|s2]>"
  Reshape_773/1 -> SignalFilter/773
  SensorOutput2/4 -> Reshape_774/1  "<a_Object_CoorSys_S[x;y;z][m|s2]>"
  Reshape_774/1 -> SignalFilter/774
  SensorOutput2/5 -> Reshape_775/1  "<Dist_Object[m]>"
  Reshape_775/1 -> SignalFilter/775
  SensorOutput2/6 -> Reshape_776/1  "<Angle_Hor_Object[deg]>"
  Reshape_776/1 -> SignalFilter/776
  SensorOutput2/7 -> Reshape_777/1  "<Angle_Ver_Object[deg]>"
  Reshape_777/1 -> SignalFilter/777
  SensorOutput2/8 -> Reshape_778/1  "<Pos_Sensor_Apex_E[x;y;z][m]>"
  Reshape_778/1 -> SignalFilter/778
  SensorOutput2/9 -> Reshape_779/1  "<Pos_Object_NearestPnt_S[x;y;z][m]>"
  Reshape_779/1 -> SignalFilter/779
  SensorOutput2/10 -> Reshape_780/1  "<Pos_Object_NearestPnt_E[x;y;z][m]>"
  Reshape_780/1 -> SignalFilter/780
  SensorOutput2/11 -> Reshape_781/1  "<Object_Info[-1None|1Fellow|2Static]>"
  Reshape_781/1 -> SignalFilter/781
  SensorOutput2/12 -> Reshape_782/1  "<Object_ID[]>"
  Reshape_782/1 -> SignalFilter/782
  SensorOutput2/13 -> Reshape_783/1  "<Object_Type[]>"
  Reshape_783/1 -> SignalFilter/783
  SensorOutput2/14 -> Reshape_784/1  "<Object_Age[s]>"
  Reshape_784/1 -> SignalFilter/784
  SensorOutput2/15 -> Reshape_785/1  "<Object_In_Scope_Entry_First[s]>"
  Reshape_785/1 -> SignalFilter/785
  SensorOutput2/16 -> Reshape_786/1  "<Object_In_Scope_Entry_Number[]>"
  Reshape_786/1 -> SignalFilter/786
  SensorOutput2/17 -> Reshape_787/1  "<Occlusion_Ratio_Object[-1|0_1]>"
  Reshape_787/1 -> SignalFilter/787
  SensorOutput2/18 -> Reshape_788/1  "<Flag_NearestPnt_Occluded[-1|0|1]>"
  Reshape_788/1 -> SignalFilter/788
  SensorOutput2/19 -> Reshape_789/1  "<Pos_NearestSurf_Pnt1_CoorSys_S[x;y;z][m]>"
  Reshape_789/1 -> SignalFilter/789
  SensorOutput2/20 -> Reshape_790/1  "<Pos_NearestSurf_Pnt2_CoorSys_S[x;y;z][m]>"
  Reshape_790/1 -> SignalFilter/790
  SensorOutput2/21 -> Reshape_791/1  "<Pos_NearestSurf_Pnt3_CoorSys_S[x;y;z][m]>"
  Reshape_791/1 -> SignalFilter/791
  SensorOutput2/22 -> Reshape_792/1  "<Pos_NearestSurf_Pnt4_CoorSys_S[x;y;z][m]>"
  Reshape_792/1 -> SignalFilter/792
  SensorOutput2/23 -> Reshape_793/1  "<NearestSurf_Pnts_Index[]>"
  Reshape_793/1 -> SignalFilter/793
  SensorOutput2/24 -> Reshape_794/1  "<NearestSurf_Index[]>"
  Reshape_794/1 -> SignalFilter/794
  SensorTimeStamp1/1 -> SignalFilter/795  "<ObjectSample[s]>"
  SensorTimeStamp1/2 -> SignalFilter/796  "<SensorCalculation[s]>"
  RadarEffects1/1 -> Reshape_797/1  "<ID[]>"
  Reshape_797/1 -> SignalFilter/797
  RadarEffects1/2 -> Reshape_798/1  "<Object_ID[]>"
  Reshape_798/1 -> SignalFilter/798
  RadarEffects1/3 -> Reshape_799/1  "<Dist_CoorSys_S[m]>"
  Reshape_799/1 -> SignalFilter/799
  RadarEffects1/4 -> Reshape_800/1  "<Angle_Hor_CoorSys_S[deg]>"
  Reshape_800/1 -> SignalFilter/800
  RadarEffects1/5 -> Reshape_801/1  "<Pos_ObjectPoint_CoorSys_E[x;y;z][m]>"
  Reshape_801/1 -> SignalFilter/801
  CustomPoints1/1 -> Reshape_802/1  "<ID[]>"
  Reshape_802/1 -> SignalFilter/802
  CustomPoints1/2 -> Reshape_803/1  "<Object_ID[]>"
  Reshape_803/1 -> SignalFilter/803
  CustomPoints1/3 -> Reshape_804/1  "<Dist_CoorSys_S[m]>"
  Reshape_804/1 -> SignalFilter/804
  CustomPoints1/4 -> Reshape_805/1  "<Angle_Hor_CoorSys_S[deg]>"
  Reshape_805/1 -> SignalFilter/805
  CustomPoints1/5 -> Reshape_806/1  "<Pos_CoorSys_E[x;y;z][m]>"
  Reshape_806/1 -> SignalFilter/806
  Object_Positions1/1 -> Reshape_807/1  "<Pos_x_MainPnt_Objects_CoorSysE[m]>"
  Reshape_807/1 -> SignalFilter/807
  Object_Positions1/2 -> Reshape_808/1  "<Pos_y_MainPnt_Objects_CoorSysE[m]>"
  Reshape_808/1 -> SignalFilter/808
  Object_Positions1/3 -> Reshape_809/1  "<Pos_z_MainPnt_Objects_CoorSysE[m]>"
  Reshape_809/1 -> SignalFilter/809
  Object_Positions1/4 -> Reshape_810/1  "<Angle_x_Objects_CoorSysE[deg]>"
  Reshape_810/1 -> SignalFilter/810
  Object_Positions1/5 -> Reshape_811/1  "<Angle_y_Objects_CoorSysE[deg]>"
  Reshape_811/1 -> SignalFilter/811
  Object_Positions1/6 -> Reshape_812/1  "<Angle_z_Objects_CoorSysE[deg]>"
  Reshape_812/1 -> SignalFilter/812
  Object_Positions1/7 -> Reshape_813/1  "<Network_Item_Type[]>"
  Reshape_813/1 -> SignalFilter/813
  Object_Positions1/8 -> Reshape_814/1  "<Network_Item_Id[]>"
  Reshape_814/1 -> SignalFilter/814
  Object_Positions1/9 -> Reshape_815/1  "<Object_ID[]>"
  Reshape_815/1 -> SignalFilter/815
  Object_Properties_Box1/1 -> Reshape_816/1  "<Flag_BoxProperties[0|1]>"
  Reshape_816/1 -> SignalFilter/816
  Object_Properties_Box1/2 -> Reshape_817/1  "<PosVec_x_CenterPnt_Object[m]>"
  Reshape_817/1 -> SignalFilter/817
  Object_Properties_Box1/3 -> Reshape_818/1  "<PosVec_y_CenterPnt_Object[m]>"
  Reshape_818/1 -> SignalFilter/818
  Object_Properties_Box1/4 -> Reshape_819/1  "<PosVec_z_CenterPnt_Object[m]>"
  Reshape_819/1 -> SignalFilter/819
  Object_Properties_Box1/5 -> Reshape_820/1  "<Length_Object[m]>"
  Reshape_820/1 -> SignalFilter/820
  Object_Properties_Box1/6 -> Reshape_821/1  "<Width_Object[m]>"
  Reshape_821/1 -> SignalFilter/821
  Object_Properties_Box1/7 -> Reshape_822/1  "<Height_Object[m]>"
  Reshape_822/1 -> SignalFilter/822
  Object_Properties_Box1/8 -> Reshape_823/1  "<Object_Type[]>"
  Reshape_823/1 -> SignalFilter/823
  Object_Custom_Values1/1 -> Reshape_824/1  "<Object_Valid[0|1]>"
  Reshape_824/1 -> SignalFilter/824
  Object_Custom_Values1/2 -> Reshape_825/1  "<CustomValues[]>"
  Reshape_825/1 -> SignalFilter/825
  Parameters3/1 -> SignalFilter/826  "<Sensor_Enable[0Off|1On]>"
  Parameters3/2 -> SignalFilter/827  "<SensorIdx[]>"
  Parameters3/3 -> SignalFilter/828  "<t_Offs_Sensor[s]>"
  Parameters3/4 -> SignalFilter/829  "<t_Cycle_Sensor[s]>"
  Parameters3/5 -> SignalFilter/830  "<t_Delay_SensorOutput[s]>"
  Parameters3/6 -> Reshape_831/1  "<Pos_Sensor_Apex_CoorSys_V[x;y;z][m]>"
  Reshape_831/1 -> SignalFilter/831
  Parameters3/7 -> SignalFilter/832  "<Angle_z_Orientation_Sensor_CoorSys_V[deg]>"
  Parameters3/8 -> SignalFilter/833  "<Angle_ScopeZone_Horizontal[deg]>"
  Parameters3/9 -> SignalFilter/834  "<Length_ScopeZone[m]>"
  Parameters3/10 -> SignalFilter/835  "<Num_SensorRays_Used[]>"
  Parameters3/11 -> SignalFilter/836  "<Sensor_Detection_Mode[1Ray|2Sector]>"
  Parameters3/12 -> SignalFilter/837  "<Object_Detection_Mode[1Object|2Continuous|3All]>"
  SensorIndex2/1 -> SignalFilter/838  "<Idx_Sensor[]>"
  SensorStatus/1 -> SignalFilter/839  "<Flag_Object_In_Scope[0Out|1In]>"
  SensorStatus/2 -> SignalFilter/840  "<Flag_Sensor_Apex_In_Object[0Out|1In]>"
  SensorOutput3/1 -> Reshape_841/1  "<Angle_Hor_Rel[deg]>"
  Reshape_841/1 -> SignalFilter/841
  SensorOutput3/2 -> Reshape_842/1  "<Object_ID[]>"
  Reshape_842/1 -> SignalFilter/842
  SensorOutput3/3 -> Reshape_843/1  "<Object_Type[]>"
  Reshape_843/1 -> SignalFilter/843
  SensorOutput3/4 -> Reshape_844/1  "<Distance[m]>"
  Reshape_844/1 -> SignalFilter/844
  SensorOutput3/5 -> Reshape_845/1  "<v_Rel[m|s]>"
  Reshape_845/1 -> SignalFilter/845
  SensorOutput3/6 -> Reshape_846/1  "<a_Rel[m|s2]>"
  Reshape_846/1 -> SignalFilter/846
  SensorOutput3/7 -> Reshape_847/1  "<Height_Min[m]>"
  Reshape_847/1 -> SignalFilter/847
  SensorOutput3/8 -> Reshape_848/1  "<Height_Max[m]>"
  Reshape_848/1 -> SignalFilter/848
  Info8/1 -> SignalFilter/849  "<ObjectSensor2D_Sfcn_State[]>"
  Info8/2 -> SignalFilter/850  "<ObjectSensor2D_Data_Valid[0|1]>"
  Info8/3 -> SignalFilter/851  "<Flag_Sensor_Init_Ready[0|1]>"
  Object_Positions2/1 -> Reshape_852/1  "<Pos_x_MainPnt_Objects_CoorSysE[m]>"
  Reshape_852/1 -> SignalFilter/852
  Object_Positions2/2 -> Reshape_853/1  "<Pos_y_MainPnt_Objects_CoorSysE[m]>"
  Reshape_853/1 -> SignalFilter/853
  Object_Positions2/3 -> Reshape_854/1  "<Pos_z_MainPnt_Objects_CoorSysE[m]>"
  Reshape_854/1 -> SignalFilter/854
  Object_Positions2/4 -> Reshape_855/1  "<Angle_x_Objects_CoorSysE[deg]>"
  Reshape_855/1 -> SignalFilter/855
  Object_Positions2/5 -> Reshape_856/1  "<Angle_y_Objects_CoorSysE[deg]>"
  Reshape_856/1 -> SignalFilter/856
  Object_Positions2/6 -> Reshape_857/1  "<Angle_z_Objects_CoorSysE[deg]>"
  Reshape_857/1 -> SignalFilter/857
  Object_Positions2/7 -> Reshape_858/1  "<Network_Item_Type[]>"
  Reshape_858/1 -> SignalFilter/858
  Object_Positions2/8 -> Reshape_859/1  "<Network_Item_Id[]>"
  Reshape_859/1 -> SignalFilter/859
  Object_Positions2/9 -> Reshape_860/1  "<Object_ID[]>"
  Reshape_860/1 -> SignalFilter/860
  Object_Properties_Box2/1 -> Reshape_861/1  "<Flag_BoxProperties[0|1]>"
  Reshape_861/1 -> SignalFilter/861
  Object_Properties_Box2/2 -> Reshape_862/1  "<PosVec_x_CenterPnt_Object[m]>"
  Reshape_862/1 -> SignalFilter/862
  Object_Properties_Box2/3 -> Reshape_863/1  "<PosVec_y_CenterPnt_Object[m]>"
  Reshape_863/1 -> SignalFilter/863
  Object_Properties_Box2/4 -> Reshape_864/1  "<PosVec_z_CenterPnt_Object[m]>"
  Reshape_864/1 -> SignalFilter/864
  Object_Properties_Box2/5 -> Reshape_865/1  "<Length_Object[m]>"
  Reshape_865/1 -> SignalFilter/865
  Object_Properties_Box2/6 -> Reshape_866/1  "<Width_Object[m]>"
  Reshape_866/1 -> SignalFilter/866
  Object_Properties_Box2/7 -> Reshape_867/1  "<Height_Object[m]>"
  Reshape_867/1 -> SignalFilter/867
  Object_Properties_Box2/8 -> Reshape_868/1  "<Object_Type[]>"
  Reshape_868/1 -> SignalFilter/868
  Object_Custom_Values2/1 -> Reshape_869/1  "<Object_Valid[0|1]>"
  Reshape_869/1 -> SignalFilter/869
  Object_Custom_Values2/2 -> Reshape_870/1  "<CustomValues[]>"
  Reshape_870/1 -> SignalFilter/870
  SignalFilter/1 -> SignalFilterGain/1
  SignalFilterGain/1 -> MDLD_DATA_CAPTURE/1
